simulink model "StarshipSystemModel"  (R2025b)
settings: Solver=VariableStepAuto  StartTime=0.0  StopTime=10.0  RelTol=1e-3
model workspace (MAT data in the model file):
  ActiveGNCMode = Simulink.Bus
  ActiveGNCMode.Alignment = -1
  ActiveGNCMode.PreserveElementDimensions = 0
  ActiveGNCMode.Elements_internal(1) = Simulink.BusElement
  ActiveGNCMode.Elements_internal(1).DimensionsMode = 'Fixed'
  ActiveGNCMode.Elements_internal(1).SamplingMode = 'Sample based'
  ActiveGNCMode.Elements_internal(1).SampleTime = -1
  ActiveGNCMode.Elements_internal(1).Name = 'stageID'
  ActiveGNCMode.Elements_internal(1).DataType_internal = 'uint8'
  ActiveGNCMode.Elements_internal(1).Complexity = 'real'
  ActiveGNCMode.Elements_internal(1).Dimensions = 1
  ActiveGNCMode.Elements_internal(2) = Simulink.BusElement
  ActiveGNCMode.Elements_internal(2).DimensionsMode = 'Fixed'
  ActiveGNCMode.Elements_internal(2).SamplingMode = 'Sample based'
  ActiveGNCMode.Elements_internal(2).SampleTime = -1
  ActiveGNCMode.Elements_internal(2).Name = 'phaseID'
  ActiveGNCMode.Elements_internal(2).DataType_internal = 'uint8'
  ActiveGNCMode.Elements_internal(2).Complexity = 'real'
  ActiveGNCMode.Elements_internal(2).Dimensions = 1
  ActiveGNCMode.Elements_internal(3) = Simulink.BusElement
  ActiveGNCMode.Elements_internal(3).DimensionsMode = 'Fixed'
  ActiveGNCMode.Elements_internal(3).SamplingMode = 'Sample based'
  ActiveGNCMode.Elements_internal(3).SampleTime = -1
  ActiveGNCMode.Elements_internal(3).Name = 'modeID'
  ActiveGNCMode.Elements_internal(3).DataType_internal = 'uint16'
  ActiveGNCMode.Elements_internal(3).Complexity = 'real'
  ActiveGNCMode.Elements_internal(3).Dimensions = 1
  ActiveGNCMode.Elements_internal(4) = Simulink.BusElement
  ActiveGNCMode.Elements_internal(4).DimensionsMode = 'Fixed'
  ActiveGNCMode.Elements_internal(4).SamplingMode = 'Sample based'
  ActiveGNCMode.Elements_internal(4).SampleTime = -1
  ActiveGNCMode.Elements_internal(4).DocUnits = 's'
  ActiveGNCMode.Elements_internal(4).Name = 'timestamp'
  ActiveGNCMode.Elements_internal(4).DataType_internal = 'double'
  ActiveGNCMode.Elements_internal(4).Complexity = 'real'
  ActiveGNCMode.Elements_internal(4).Dimensions = 1
  ActiveGNCMode.DataScope = 'Auto'
  AerodynamicControlCommand = Simulink.Bus
  AerodynamicControlCommand.Alignment = -1
  AerodynamicControlCommand.PreserveElementDimensions = 0
  AerodynamicControlCommand.Elements_internal(1) = Simulink.BusElement
  AerodynamicControlCommand.Elements_internal(1).DimensionsMode = 'Fixed'
  AerodynamicControlCommand.Elements_internal(1).SamplingMode = 'Sample based'
  AerodynamicControlCommand.Elements_internal(1).SampleTime = -1
  AerodynamicControlCommand.Elements_internal(1).DocUnits = 'rad'
  AerodynamicControlCommand.Elements_internal(1).Name = 'surfaceCommand'
  AerodynamicControlCommand.Elements_internal(1).DataType_internal = 'double'
  AerodynamicControlCommand.Elements_internal(1).Complexity = 'real'
  AerodynamicControlCommand.Elements_internal(1).Dimensions = 1
  AerodynamicControlCommand.Elements_internal(2) = Simulink.BusElement
  AerodynamicControlCommand.Elements_internal(2).DimensionsMode = 'Fixed'
  AerodynamicControlCommand.Elements_internal(2).SamplingMode = 'Sample based'
  AerodynamicControlCommand.Elements_internal(2).SampleTime = -1
  AerodynamicControlCommand.Elements_internal(2).Name = 'mode'
  AerodynamicControlCommand.Elements_internal(2).DataType_internal = 'enum'
  AerodynamicControlCommand.Elements_internal(2).Complexity = 'real'
  AerodynamicControlCommand.Elements_internal(2).Dimensions = 1
  AerodynamicControlCommand.Elements_internal(3) = Simulink.BusElement
  AerodynamicControlCommand.Elements_internal(3).DimensionsMode = 'Fixed'
  AerodynamicControlCommand.Elements_internal(3).SamplingMode = 'Sample based'
  AerodynamicControlCommand.Elements_internal(3).SampleTime = -1
  AerodynamicControlCommand.Elements_internal(3).Name = 'enable'
  AerodynamicControlCommand.Elements_internal(3).DataType_internal = 'boolean'
  AerodynamicControlCommand.Elements_internal(3).Complexity = 'real'
  AerodynamicControlCommand.Elements_internal(3).Dimensions = 1
  AerodynamicControlCommand.Elements_internal(4) = Simulink.BusElement
  AerodynamicControlCommand.Elements_internal(4).DimensionsMode = 'Fixed'
  AerodynamicControlCommand.Elements_internal(4).SamplingMode = 'Sample based'
  AerodynamicControlCommand.Elements_internal(4).SampleTime = -1
  AerodynamicControlCommand.Elements_internal(4).Name = 'validity'
  AerodynamicControlCommand.Elements_internal(4).DataType_internal = 'enum'
  AerodynamicControlCommand.Elements_internal(4).Complexity = 'real'
  AerodynamicControlCommand.Elements_internal(4).Dimensions = 1
  AerodynamicControlCommand.Elements_internal(5) = Simulink.BusElement
  AerodynamicControlCommand.Elements_internal(5).DimensionsMode = 'Fixed'
  AerodynamicControlCommand.Elements_internal(5).SamplingMode = 'Sample based'
  AerodynamicControlCommand.Elements_internal(5).SampleTime = -1
  AerodynamicControlCommand.Elements_internal(5).DocUnits = 's'
  AerodynamicControlCommand.Elements_internal(5).Name = 'timestamp'
  AerodynamicControlCommand.Elements_internal(5).DataType_internal = 'double'
  AerodynamicControlCommand.Elements_internal(5).Complexity = 'real'
  AerodynamicControlCommand.Elements_internal(5).Dimensions = 1
  AerodynamicControlCommand.DataScope = 'Auto'
  AerodynamicLoad = Simulink.Bus
  AerodynamicLoad.Alignment = -1
  AerodynamicLoad.PreserveElementDimensions = 0
  AerodynamicLoad.Elements_internal(1) = Simulink.BusElement
  AerodynamicLoad.Elements_internal(1).DimensionsMode = 'Fixed'
  AerodynamicLoad.Elements_internal(1).SamplingMode = 'Sample based'
  AerodynamicLoad.Elements_internal(1).SampleTime = -1
  AerodynamicLoad.Elements_internal(1).DocUnits = 'N'
  AerodynamicLoad.Elements_internal(1).Name = 'force'
  AerodynamicLoad.Elements_internal(1).DataType_internal = 'double'
  AerodynamicLoad.Elements_internal(1).Complexity = 'real'
  AerodynamicLoad.Elements_internal(1).Dimensions = 1
  AerodynamicLoad.Elements_internal(2) = Simulink.BusElement
  AerodynamicLoad.Elements_internal(2).DimensionsMode = 'Fixed'
  AerodynamicLoad.Elements_internal(2).SamplingMode = 'Sample based'
  AerodynamicLoad.Elements_internal(2).SampleTime = -1
  AerodynamicLoad.Elements_internal(2).DocUnits = 'N·m'
  AerodynamicLoad.Elements_internal(2).Name = 'moment'
  AerodynamicLoad.Elements_internal(2).DataType_internal = 'double'
  AerodynamicLoad.Elements_internal(2).Complexity = 'real'
  AerodynamicLoad.Elements_internal(2).Dimensions = 1
  AerodynamicLoad.Elements_internal(3) = Simulink.BusElement
  AerodynamicLoad.Elements_internal(3).DimensionsMode = 'Fixed'
  AerodynamicLoad.Elements_internal(3).SamplingMode = 'Sample based'
  AerodynamicLoad.Elements_internal(3).SampleTime = -1
  AerodynamicLoad.Elements_internal(3).Name = 'referenceFrame'
  AerodynamicLoad.Elements_internal(3).DataType_internal = 'string'
  AerodynamicLoad.Elements_internal(3).Complexity = 'real'
  AerodynamicLoad.Elements_internal(3).Dimensions = 1
  AerodynamicLoad.Elements_internal(4) = Simulink.BusElement
  AerodynamicLoad.Elements_internal(4).DimensionsMode = 'Fixed'
  AerodynamicLoad.Elements_internal(4).SamplingMode = 'Sample based'
  AerodynamicLoad.Elements_internal(4).SampleTime = -1
  AerodynamicLoad.Elements_internal(4).DocUnits = 'Pa'
  AerodynamicLoad.Elements_internal(4).Name = 'surfacePressure'
  AerodynamicLoad.Elements_internal(4).DataType_internal = 'double'
  AerodynamicLoad.Elements_internal(4).Complexity = 'real'
  AerodynamicLoad.Elements_internal(4).Dimensions = 1
  AerodynamicLoad.Elements_internal(5) = Simulink.BusElement
  AerodynamicLoad.Elements_internal(5).DimensionsMode = 'Fixed'
  AerodynamicLoad.Elements_internal(5).SamplingMode = 'Sample based'
  AerodynamicLoad.Elements_internal(5).SampleTime = -1
  AerodynamicLoad.Elements_internal(5).Name = 'validity'
  AerodynamicLoad.Elements_internal(5).DataType_internal = 'enum'
  AerodynamicLoad.Elements_internal(5).Complexity = 'real'
  AerodynamicLoad.Elements_internal(5).Dimensions = 1
  AerodynamicLoad.DataScope = 'Auto'
  AggregatedStream = Simulink.Bus
  AggregatedStream.Alignment = -1
  AggregatedStream.PreserveElementDimensions = 0
  AggregatedStream.Elements_internal(1) = Simulink.BusElement
  AggregatedStream.Elements_internal(1).DimensionsMode = 'Fixed'
  AggregatedStream.Elements_internal(1).SamplingMode = 'Sample based'
  AggregatedStream.Elements_internal(1).SampleTime = -1
  AggregatedStream.Elements_internal(1).Name = 'payload'
  AggregatedStream.Elements_internal(1).DataType_internal = 'uint8'
  AggregatedStream.Elements_internal(1).Complexity = 'real'
  AggregatedStream.Elements_internal(1).Dimensions = 1
  AggregatedStream.Elements_internal(2) = Simulink.BusElement
  AggregatedStream.Elements_internal(2).DimensionsMode = 'Fixed'
  AggregatedStream.Elements_internal(2).SamplingMode = 'Sample based'
  AggregatedStream.Elements_internal(2).SampleTime = -1
  AggregatedStream.Elements_internal(2).Name = 'sourceMix'
  AggregatedStream.Elements_internal(2).DataType_internal = 'double'
  AggregatedStream.Elements_internal(2).Complexity = 'real'
  AggregatedStream.Elements_internal(2).Dimensions = 1
  AggregatedStream.Elements_internal(3) = Simulink.BusElement
  AggregatedStream.Elements_internal(3).DimensionsMode = 'Fixed'
  AggregatedStream.Elements_internal(3).SamplingMode = 'Sample based'
  AggregatedStream.Elements_internal(3).SampleTime = -1
  AggregatedStream.Elements_internal(3).DocUnits = 's'
  AggregatedStream.Elements_internal(3).Name = 'timestamp'
  AggregatedStream.Elements_internal(3).DataType_internal = 'double'
  AggregatedStream.Elements_internal(3).Complexity = 'real'
  AggregatedStream.Elements_internal(3).Dimensions = 1
  AggregatedStream.DataScope = 'Auto'
  AllocatedEffectorDemand = Simulink.Bus
  AllocatedEffectorDemand.Alignment = -1
  AllocatedEffectorDemand.PreserveElementDimensions = 0
  AllocatedEffectorDemand.Elements_internal(1) = Simulink.BusElement
  AllocatedEffectorDemand.Elements_internal(1).DimensionsMode = 'Fixed'
  AllocatedEffectorDemand.Elements_internal(1).SamplingMode = 'Sample based'
  AllocatedEffectorDemand.Elements_internal(1).SampleTime = -1
  AllocatedEffectorDemand.Elements_internal(1).Name = 'effectorID'
  AllocatedEffectorDemand.Elements_internal(1).DataType_internal = 'uint16'
  AllocatedEffectorDemand.Elements_internal(1).Complexity = 'real'
  AllocatedEffectorDemand.Elements_internal(1).Dimensions = 1
  AllocatedEffectorDemand.Elements_internal(2) = Simulink.BusElement
  AllocatedEffectorDemand.Elements_internal(2).DimensionsMode = 'Fixed'
  AllocatedEffectorDemand.Elements_internal(2).SamplingMode = 'Sample based'
  AllocatedEffectorDemand.Elements_internal(2).SampleTime = -1
  AllocatedEffectorDemand.Elements_internal(2).Name = 'demand'
  AllocatedEffectorDemand.Elements_internal(2).DataType_internal = 'double'
  AllocatedEffectorDemand.Elements_internal(2).Complexity = 'real'
  AllocatedEffectorDemand.Elements_internal(2).Dimensions = 1
  AllocatedEffectorDemand.Elements_internal(3) = Simulink.BusElement
  AllocatedEffectorDemand.Elements_internal(3).DimensionsMode = 'Fixed'
  AllocatedEffectorDemand.Elements_internal(3).SamplingMode = 'Sample based'
  AllocatedEffectorDemand.Elements_internal(3).SampleTime = -1
  AllocatedEffectorDemand.Elements_internal(3).Name = 'validity'
  AllocatedEffectorDemand.Elements_internal(3).DataType_internal = 'uint8'
  AllocatedEffectorDemand.Elements_internal(3).Complexity = 'real'
  AllocatedEffectorDemand.Elements_internal(3).Dimensions = 1
  AllocatedEffectorDemand.Elements_internal(4) = Simulink.BusElement
  AllocatedEffectorDemand.Elements_internal(4).DimensionsMode = 'Fixed'
  AllocatedEffectorDemand.Elements_internal(4).SamplingMode = 'Sample based'
  AllocatedEffectorDemand.Elements_internal(4).SampleTime = -1
  AllocatedEffectorDemand.Elements_internal(4).DocUnits = 's'
  AllocatedEffectorDemand.Elements_internal(4).Name = 'timestamp'
  AllocatedEffectorDemand.Elements_internal(4).DataType_internal = 'double'
  AllocatedEffectorDemand.Elements_internal(4).Complexity = 'real'
  AllocatedEffectorDemand.Elements_internal(4).Dimensions = 1
  AllocatedEffectorDemand.DataScope = 'Auto'
  AttitudeControlDemand = Simulink.Bus
  AttitudeControlDemand.Alignment = -1
  AttitudeControlDemand.PreserveElementDimensions = 0
  AttitudeControlDemand.Elements_internal(1) = Simulink.BusElement
  AttitudeControlDemand.Elements_internal(1).DimensionsMode = 'Fixed'
  AttitudeControlDemand.Elements_internal(1).SamplingMode = 'Sample based'
  AttitudeControlDemand.Elements_internal(1).SampleTime = -1
  AttitudeControlDemand.Elements_internal(1).DocUnits = 'N.m'
  AttitudeControlDemand.Elements_internal(1).Name = 'torqueDemand'
  AttitudeControlDemand.Elements_internal(1).DataType_internal = 'double'
  AttitudeControlDemand.Elements_internal(1).Complexity = 'real'
  AttitudeControlDemand.Elements_internal(1).Dimensions = 3
  AttitudeControlDemand.Elements_internal(2) = Simulink.BusElement
  AttitudeControlDemand.Elements_internal(2).DimensionsMode = 'Fixed'
  AttitudeControlDemand.Elements_internal(2).SamplingMode = 'Sample based'
  AttitudeControlDemand.Elements_internal(2).SampleTime = -1
  AttitudeControlDemand.Elements_internal(2).DocUnits = 's'
  AttitudeControlDemand.Elements_internal(2).Name = 'timestamp'
  AttitudeControlDemand.Elements_internal(2).DataType_internal = 'double'
  AttitudeControlDemand.Elements_internal(2).Complexity = 'real'
  AttitudeControlDemand.Elements_internal(2).Dimensions = 1
  AttitudeControlDemand.DataScope = 'Auto'
  AttitudeGuidanceCommand = Simulink.Bus
  AttitudeGuidanceCommand.Alignment = -1
  AttitudeGuidanceCommand.PreserveElementDimensions = 0
  AttitudeGuidanceCommand.Elements_internal(1) = Simulink.BusElement
  AttitudeGuidanceCommand.Elements_internal(1).DimensionsMode = 'Fixed'
  AttitudeGuidanceCommand.Elements_internal(1).SamplingMode = 'Sample based'
  AttitudeGuidanceCommand.Elements_internal(1).SampleTime = -1
  AttitudeGuidanceCommand.Elements_internal(1).Name = 'attitudeTarget'
  AttitudeGuidanceCommand.Elements_internal(1).DataType_internal = 'double'
  AttitudeGuidanceCommand.Elements_internal(1).Complexity = 'real'
  AttitudeGuidanceCommand.Elements_internal(1).Dimensions = 4
  AttitudeGuidanceCommand.Elements_internal(2) = Simulink.BusElement
  AttitudeGuidanceCommand.Elements_internal(2).DimensionsMode = 'Fixed'
  AttitudeGuidanceCommand.Elements_internal(2).SamplingMode = 'Sample based'
  AttitudeGuidanceCommand.Elements_internal(2).SampleTime = -1
  AttitudeGuidanceCommand.Elements_internal(2).Name = 'rateTarget'
  AttitudeGuidanceCommand.Elements_internal(2).DataType_internal = 'double'
  AttitudeGuidanceCommand.Elements_internal(2).Complexity = 'real'
  AttitudeGuidanceCommand.Elements_internal(2).Dimensions = 3
  AttitudeGuidanceCommand.Elements_internal(3) = Simulink.BusElement
  AttitudeGuidanceCommand.Elements_internal(3).DimensionsMode = 'Fixed'
  AttitudeGuidanceCommand.Elements_internal(3).SamplingMode = 'Sample based'
  AttitudeGuidanceCommand.Elements_internal(3).SampleTime = -1
  AttitudeGuidanceCommand.Elements_internal(3).DocUnits = 's'
  AttitudeGuidanceCommand.Elements_internal(3).Name = 'timestamp'
  AttitudeGuidanceCommand.Elements_internal(3).DataType_internal = 'double'
  AttitudeGuidanceCommand.Elements_internal(3).Complexity = 'real'
  AttitudeGuidanceCommand.Elements_internal(3).Dimensions = 1
  AttitudeGuidanceCommand.DataScope = 'Auto'
  AttitudeRateState = Simulink.Bus
  AttitudeRateState.Alignment = -1
  AttitudeRateState.PreserveElementDimensions = 0
  AttitudeRateState.Elements_internal(1) = Simulink.BusElement
  AttitudeRateState.Elements_internal(1).DimensionsMode = 'Fixed'
  AttitudeRateState.Elements_internal(1).SamplingMode = 'Sample based'
  AttitudeRateState.Elements_internal(1).SampleTime = -1
  AttitudeRateState.Elements_internal(1).Name = 'attitude'
  AttitudeRateState.Elements_internal(1).DataType_internal = 'double'
  AttitudeRateState.Elements_internal(1).Complexity = 'real'
  AttitudeRateState.Elements_internal(1).Dimensions = 4
  AttitudeRateState.Elements_internal(2) = Simulink.BusElement
  AttitudeRateState.Elements_internal(2).DimensionsMode = 'Fixed'
  AttitudeRateState.Elements_internal(2).SamplingMode = 'Sample based'
  AttitudeRateState.Elements_internal(2).SampleTime = -1
  AttitudeRateState.Elements_internal(2).DocUnits = 'rad/s'
  AttitudeRateState.Elements_internal(2).Name = 'angularRate'
  AttitudeRateState.Elements_internal(2).DataType_internal = 'double'
  AttitudeRateState.Elements_internal(2).Complexity = 'real'
  AttitudeRateState.Elements_internal(2).Dimensions = 3
  AttitudeRateState.Elements_internal(3) = Simulink.BusElement
  AttitudeRateState.Elements_internal(3).DimensionsMode = 'Fixed'
  AttitudeRateState.Elements_internal(3).SamplingMode = 'Sample based'
  AttitudeRateState.Elements_internal(3).SampleTime = -1
  AttitudeRateState.Elements_internal(3).DocUnits = 's'
  AttitudeRateState.Elements_internal(3).Name = 'timestamp'
  AttitudeRateState.Elements_internal(3).DataType_internal = 'double'
  AttitudeRateState.Elements_internal(3).Complexity = 'real'
  AttitudeRateState.Elements_internal(3).Dimensions = 1
  AttitudeRateState.DataScope = 'Auto'
  AutogenousPressurantGas = Simulink.ConnectionBus
  AutogenousPressurantGas.Elements_internal = Simulink.ConnectionElement
  AutogenousPressurantGas.Elements_internal.Name = 'Element'
  AutogenousPressurantGas.Elements_internal.Type_internal = 'Connection: foundation.gas.gas'
  CandidateFaultIndication = Simulink.Bus
  CandidateFaultIndication.Alignment = -1
  CandidateFaultIndication.PreserveElementDimensions = 0
  CandidateFaultIndication.Elements_internal(1) = Simulink.BusElement
  CandidateFaultIndication.Elements_internal(1).DimensionsMode = 'Fixed'
  CandidateFaultIndication.Elements_internal(1).SamplingMode = 'Sample based'
  CandidateFaultIndication.Elements_internal(1).SampleTime = -1
  CandidateFaultIndication.Elements_internal(1).Name = 'faultCode'
  CandidateFaultIndication.Elements_internal(1).DataType_internal = 'string'
  CandidateFaultIndication.Elements_internal(1).Complexity = 'real'
  CandidateFaultIndication.Elements_internal(1).Dimensions = 1
  CandidateFaultIndication.Elements_internal(2) = Simulink.BusElement
  CandidateFaultIndication.Elements_internal(2).DimensionsMode = 'Fixed'
  CandidateFaultIndication.Elements_internal(2).SamplingMode = 'Sample based'
  CandidateFaultIndication.Elements_internal(2).SampleTime = -1
  CandidateFaultIndication.Elements_internal(2).Name = 'confidence'
  CandidateFaultIndication.Elements_internal(2).DataType_internal = 'string'
  CandidateFaultIndication.Elements_internal(2).Complexity = 'real'
  CandidateFaultIndication.Elements_internal(2).Dimensions = 1
  CandidateFaultIndication.DataScope = 'Auto'
  CombustionGasFeed = Simulink.ConnectionBus
  CombustionGasFeed.Elements_internal = Simulink.ConnectionElement
  CombustionGasFeed.Elements_internal.Name = 'Element'
  CombustionGasFeed.Elements_internal.Type_internal = 'Connection: foundation.gas.gas'
  CommandPathHealth = Simulink.Bus
  CommandPathHealth.Alignment = -1
  CommandPathHealth.PreserveElementDimensions = 0
  CommandPathHealth.Elements_internal(1) = Simulink.BusElement
  CommandPathHealth.Elements_internal(1).DimensionsMode = 'Fixed'
  CommandPathHealth.Elements_internal(1).SamplingMode = 'Sample based'
  CommandPathHealth.Elements_internal(1).SampleTime = -1
  CommandPathHealth.Elements_internal(1).Name = 'availability'
  CommandPathHealth.Elements_internal(1).DataType_internal = 'uint8'
  CommandPathHealth.Elements_internal(1).Complexity = 'real'
  CommandPathHealth.Elements_internal(1).Dimensions = 1
  CommandPathHealth.Elements_internal(2) = Simulink.BusElement
  CommandPathHealth.Elements_internal(2).DimensionsMode = 'Fixed'
  CommandPathHealth.Elements_internal(2).SamplingMode = 'Sample based'
  CommandPathHealth.Elements_internal(2).SampleTime = -1
  CommandPathHealth.Elements_internal(2).Name = 'inhibitedReason'
  CommandPathHealth.Elements_internal(2).DataType_internal = 'uint16'
  CommandPathHealth.Elements_internal(2).Complexity = 'real'
  CommandPathHealth.Elements_internal(2).Dimensions = 1
  CommandPathHealth.Elements_internal(3) = Simulink.BusElement
  CommandPathHealth.Elements_internal(3).DimensionsMode = 'Fixed'
  CommandPathHealth.Elements_internal(3).SamplingMode = 'Sample based'
  CommandPathHealth.Elements_internal(3).SampleTime = -1
  CommandPathHealth.Elements_internal(3).DocUnits = 's'
  CommandPathHealth.Elements_internal(3).Name = 'timestamp'
  CommandPathHealth.Elements_internal(3).DataType_internal = 'double'
  CommandPathHealth.Elements_internal(3).Complexity = 'real'
  CommandPathHealth.Elements_internal(3).Dimensions = 1
  CommandPathHealth.DataScope = 'Auto'
  ControlMode = Simulink.ValueType
  ControlMode.DataType = 'enum'
  DownlinkSignal = Simulink.Bus
  DownlinkSignal.Alignment = -1
  DownlinkSignal.PreserveElementDimensions = 0
  DownlinkSignal.Elements_internal(1) = Simulink.BusElement
  DownlinkSignal.Elements_internal(1).DimensionsMode = 'Fixed'
  DownlinkSignal.Elements_internal(1).SamplingMode = 'Sample based'
  DownlinkSignal.Elements_internal(1).SampleTime = -1
  DownlinkSignal.Elements_internal(1).Name = 'payload'
  DownlinkSignal.Elements_internal(1).DataType_internal = 'uint8'
  DownlinkSignal.Elements_internal(1).Complexity = 'real'
  DownlinkSignal.Elements_internal(1).Dimensions = 1
  DownlinkSignal.Elements_internal(2) = Simulink.BusElement
  DownlinkSignal.Elements_internal(2).DimensionsMode = 'Fixed'
  DownlinkSignal.Elements_internal(2).SamplingMode = 'Sample based'
  DownlinkSignal.Elements_internal(2).SampleTime = -1
  DownlinkSignal.Elements_internal(2).Description = '{Relay, DirectRF}'
  DownlinkSignal.Elements_internal(2).Name = 'pathUsed'
  DownlinkSignal.Elements_internal(2).DataType_internal = 'enumration'
  DownlinkSignal.Elements_internal(2).Complexity = 'real'
  DownlinkSignal.Elements_internal(2).Dimensions = 1
  DownlinkSignal.Elements_internal(3) = Simulink.BusElement
  DownlinkSignal.Elements_internal(3).DimensionsMode = 'Fixed'
  DownlinkSignal.Elements_internal(3).SamplingMode = 'Sample based'
  DownlinkSignal.Elements_internal(3).SampleTime = -1
  DownlinkSignal.Elements_internal(3).DocUnits = 's'
  DownlinkSignal.Elements_internal(3).Name = 'timestamp'
  DownlinkSignal.Elements_internal(3).DataType_internal = 'double'
  DownlinkSignal.Elements_internal(3).Complexity = 'real'
  DownlinkSignal.Elements_internal(3).Dimensions = 1
  DownlinkSignal.DataScope = 'Auto'
  ElectricalPower = Simulink.ConnectionBus
  ElectricalPower.Elements_internal = Simulink.ConnectionElement
  ElectricalPower.Elements_internal.Name = 'Element'
  ElectricalPower.Elements_internal.Type_internal = 'Connection: foundation.electrical.electrical'
  EngineTelemetry = Simulink.Bus
  EngineTelemetry.Alignment = -1
  EngineTelemetry.PreserveElementDimensions = 0
  EngineTelemetry.Elements_internal(1) = Simulink.BusElement
  EngineTelemetry.Elements_internal(1).DimensionsMode = 'Fixed'
  EngineTelemetry.Elements_internal(1).SamplingMode = 'Sample based'
  EngineTelemetry.Elements_internal(1).SampleTime = -1
  EngineTelemetry.Elements_internal(1).DocUnits = 'Pa'
  EngineTelemetry.Elements_internal(1).Name = 'chamberPressure'
  EngineTelemetry.Elements_internal(1).DataType_internal = 'double'
  EngineTelemetry.Elements_internal(1).Complexity = 'real'
  EngineTelemetry.Elements_internal(1).Dimensions = 1
  EngineTelemetry.Elements_internal(2) = Simulink.BusElement
  EngineTelemetry.Elements_internal(2).DimensionsMode = 'Fixed'
  EngineTelemetry.Elements_internal(2).SamplingMode = 'Sample based'
  EngineTelemetry.Elements_internal(2).SampleTime = -1
  EngineTelemetry.Elements_internal(2).DocUnits = 'rpm'
  EngineTelemetry.Elements_internal(2).Name = 'turbopumpSpeed'
  EngineTelemetry.Elements_internal(2).DataType_internal = 'double'
  EngineTelemetry.Elements_internal(2).Complexity = 'real'
  EngineTelemetry.Elements_internal(2).Dimensions = 1
  EngineTelemetry.Elements_internal(3) = Simulink.BusElement
  EngineTelemetry.Elements_internal(3).DimensionsMode = 'Fixed'
  EngineTelemetry.Elements_internal(3).SamplingMode = 'Sample based'
  EngineTelemetry.Elements_internal(3).SampleTime = -1
  EngineTelemetry.Elements_internal(3).DocUnits = 'K'
  EngineTelemetry.Elements_internal(3).Name = 'temperature'
  EngineTelemetry.Elements_internal(3).DataType_internal = 'double'
  EngineTelemetry.Elements_internal(3).Complexity = 'real'
  EngineTelemetry.Elements_internal(3).Dimensions = 1
  EngineTelemetry.Elements_internal(4) = Simulink.BusElement
  EngineTelemetry.Elements_internal(4).DimensionsMode = 'Fixed'
  EngineTelemetry.Elements_internal(4).SamplingMode = 'Sample based'
  EngineTelemetry.Elements_internal(4).SampleTime = -1
  EngineTelemetry.Elements_internal(4).Name = 'status'
  EngineTelemetry.Elements_internal(4).DataType_internal = 'uint8'
  EngineTelemetry.Elements_internal(4).Complexity = 'real'
  EngineTelemetry.Elements_internal(4).Dimensions = 1
  EngineTelemetry.DataScope = 'Auto'
  ExecutionContext = Simulink.Bus
  ExecutionContext.Alignment = -1
  ExecutionContext.PreserveElementDimensions = 0
  ExecutionContext.Elements_internal(1) = Simulink.BusElement
  ExecutionContext.Elements_internal(1).DimensionsMode = 'Fixed'
  ExecutionContext.Elements_internal(1).SamplingMode = 'Sample based'
  ExecutionContext.Elements_internal(1).SampleTime = -1
  ExecutionContext.Elements_internal(1).Name = 'cycleID'
  ExecutionContext.Elements_internal(1).DataType_internal = 'uint32'
  ExecutionContext.Elements_internal(1).Complexity = 'real'
  ExecutionContext.Elements_internal(1).Dimensions = 1
  ExecutionContext.Elements_internal(2) = Simulink.BusElement
  ExecutionContext.Elements_internal(2).DimensionsMode = 'Fixed'
  ExecutionContext.Elements_internal(2).SamplingMode = 'Sample based'
  ExecutionContext.Elements_internal(2).SampleTime = -1
  ExecutionContext.Elements_internal(2).Name = 'phaseID'
  ExecutionContext.Elements_internal(2).DataType_internal = 'uint8'
  ExecutionContext.Elements_internal(2).Complexity = 'real'
  ExecutionContext.Elements_internal(2).Dimensions = 1
  ExecutionContext.Elements_internal(3) = Simulink.BusElement
  ExecutionContext.Elements_internal(3).DimensionsMode = 'Fixed'
  ExecutionContext.Elements_internal(3).SamplingMode = 'Sample based'
  ExecutionContext.Elements_internal(3).SampleTime = -1
  ExecutionContext.Elements_internal(3).Name = 'executionStatus'
  ExecutionContext.Elements_internal(3).DataType_internal = 'uint8'
  ExecutionContext.Elements_internal(3).Complexity = 'real'
  ExecutionContext.Elements_internal(3).Dimensions = 1
  ExecutionContext.Elements_internal(4) = Simulink.BusElement
  ExecutionContext.Elements_internal(4).DimensionsMode = 'Fixed'
  ExecutionContext.Elements_internal(4).SamplingMode = 'Sample based'
  ExecutionContext.Elements_internal(4).SampleTime = -1
  ExecutionContext.Elements_internal(4).DocUnits = 's'
  ExecutionContext.Elements_internal(4).Name = 'timestamp'
  ExecutionContext.Elements_internal(4).DataType_internal = 'double'
  ExecutionContext.Elements_internal(4).Complexity = 'real'
  ExecutionContext.Elements_internal(4).Dimensions = 1
  ExecutionContext.DataScope = 'Auto'
  FaultDiagnosisResult = Simulink.Bus
  FaultDiagnosisResult.Alignment = -1
  FaultDiagnosisResult.PreserveElementDimensions = 0
  FaultDiagnosisResult.Elements_internal(1) = Simulink.BusElement
  FaultDiagnosisResult.Elements_internal(1).DimensionsMode = 'Fixed'
  FaultDiagnosisResult.Elements_internal(1).SamplingMode = 'Sample based'
  FaultDiagnosisResult.Elements_internal(1).SampleTime = -1
  FaultDiagnosisResult.Elements_internal(1).Name = 'faultCode'
  FaultDiagnosisResult.Elements_internal(1).DataType_internal = 'string'
  FaultDiagnosisResult.Elements_internal(1).Complexity = 'real'
  FaultDiagnosisResult.Elements_internal(1).Dimensions = 1
  FaultDiagnosisResult.Elements_internal(2) = Simulink.BusElement
  FaultDiagnosisResult.Elements_internal(2).DimensionsMode = 'Fixed'
  FaultDiagnosisResult.Elements_internal(2).SamplingMode = 'Sample based'
  FaultDiagnosisResult.Elements_internal(2).SampleTime = -1
  FaultDiagnosisResult.Elements_internal(2).Name = 'confidence'
  FaultDiagnosisResult.Elements_internal(2).DataType_internal = 'string'
  FaultDiagnosisResult.Elements_internal(2).Complexity = 'real'
  FaultDiagnosisResult.Elements_internal(2).Dimensions = 1
  FaultDiagnosisResult.DataScope = 'Auto'
  GNCDataContext = Simulink.Bus
  GNCDataContext.Alignment = -1
  GNCDataContext.PreserveElementDimensions = 0
  GNCDataContext.Elements_internal(1) = Simulink.BusElement
  GNCDataContext.Elements_internal(1).DimensionsMode = 'Fixed'
  GNCDataContext.Elements_internal(1).SamplingMode = 'Sample based'
  GNCDataContext.Elements_internal(1).SampleTime = -1
  GNCDataContext.Elements_internal(1).Name = 'sourceID'
  GNCDataContext.Elements_internal(1).DataType_internal = 'uint16'
  GNCDataContext.Elements_internal(1).Complexity = 'real'
  GNCDataContext.Elements_internal(1).Dimensions = 1
  GNCDataContext.Elements_internal(2) = Simulink.BusElement
  GNCDataContext.Elements_internal(2).DimensionsMode = 'Fixed'
  GNCDataContext.Elements_internal(2).SamplingMode = 'Sample based'
  GNCDataContext.Elements_internal(2).SampleTime = -1
  GNCDataContext.Elements_internal(2).Name = 'dataClass'
  GNCDataContext.Elements_internal(2).DataType_internal = 'uint8'
  GNCDataContext.Elements_internal(2).Complexity = 'real'
  GNCDataContext.Elements_internal(2).Dimensions = 1
  GNCDataContext.Elements_internal(3) = Simulink.BusElement
  GNCDataContext.Elements_internal(3).DimensionsMode = 'Fixed'
  GNCDataContext.Elements_internal(3).SamplingMode = 'Sample based'
  GNCDataContext.Elements_internal(3).SampleTime = -1
  GNCDataContext.Elements_internal(3).DocUnits = 's'
  GNCDataContext.Elements_internal(3).Name = 'timestamp'
  GNCDataContext.Elements_internal(3).DataType_internal = 'double'
  GNCDataContext.Elements_internal(3).Complexity = 'real'
  GNCDataContext.Elements_internal(3).Dimensions = 1
  GNCDataContext.Elements_internal(4) = Simulink.BusElement
  GNCDataContext.Elements_internal(4).DimensionsMode = 'Fixed'
  GNCDataContext.Elements_internal(4).SamplingMode = 'Sample based'
  GNCDataContext.Elements_internal(4).SampleTime = -1
  GNCDataContext.Elements_internal(4).Name = 'validity'
  GNCDataContext.Elements_internal(4).DataType_internal = 'uint8'
  GNCDataContext.Elements_internal(4).Complexity = 'real'
  GNCDataContext.Elements_internal(4).Dimensions = 1
  GNCDataContext.DataScope = 'Auto'
  GNCHealthState = Simulink.Bus
  GNCHealthState.Alignment = -1
  GNCHealthState.PreserveElementDimensions = 0
  GNCHealthState.Elements_internal(1) = Simulink.BusElement
  GNCHealthState.Elements_internal(1).DimensionsMode = 'Fixed'
  GNCHealthState.Elements_internal(1).SamplingMode = 'Sample based'
  GNCHealthState.Elements_internal(1).SampleTime = -1
  GNCHealthState.Elements_internal(1).Name = 'healthState'
  GNCHealthState.Elements_internal(1).DataType_internal = 'uint8'
  GNCHealthState.Elements_internal(1).Complexity = 'real'
  GNCHealthState.Elements_internal(1).Dimensions = 1
  GNCHealthState.Elements_internal(2) = Simulink.BusElement
  GNCHealthState.Elements_internal(2).DimensionsMode = 'Fixed'
  GNCHealthState.Elements_internal(2).SamplingMode = 'Sample based'
  GNCHealthState.Elements_internal(2).SampleTime = -1
  GNCHealthState.Elements_internal(2).Name = 'faultCode'
  GNCHealthState.Elements_internal(2).DataType_internal = 'uint16'
  GNCHealthState.Elements_internal(2).Complexity = 'real'
  GNCHealthState.Elements_internal(2).Dimensions = 1
  GNCHealthState.Elements_internal(3) = Simulink.BusElement
  GNCHealthState.Elements_internal(3).DimensionsMode = 'Fixed'
  GNCHealthState.Elements_internal(3).SamplingMode = 'Sample based'
  GNCHealthState.Elements_internal(3).SampleTime = -1
  GNCHealthState.Elements_internal(3).DocUnits = 's'
  GNCHealthState.Elements_internal(3).Name = 'timestamp'
  GNCHealthState.Elements_internal(3).DataType_internal = 'double'
  GNCHealthState.Elements_internal(3).Complexity = 'real'
  GNCHealthState.Elements_internal(3).Dimensions = 1
  GNCHealthState.DataScope = 'Auto'
  GNCStateEstimate = Simulink.Bus
  GNCStateEstimate.Alignment = -1
  GNCStateEstimate.PreserveElementDimensions = 0
  GNCStateEstimate.Elements_internal(1) = Simulink.BusElement
  GNCStateEstimate.Elements_internal(1).DimensionsMode = 'Fixed'
  GNCStateEstimate.Elements_internal(1).SamplingMode = 'Sample based'
  GNCStateEstimate.Elements_internal(1).SampleTime = -1
  GNCStateEstimate.Elements_internal(1).DocUnits = 'm'
  GNCStateEstimate.Elements_internal(1).Name = 'position'
  GNCStateEstimate.Elements_internal(1).DataType_internal = 'double'
  GNCStateEstimate.Elements_internal(1).Complexity = 'real'
  GNCStateEstimate.Elements_internal(1).Dimensions = 3
  GNCStateEstimate.Elements_internal(2) = Simulink.BusElement
  GNCStateEstimate.Elements_internal(2).DimensionsMode = 'Fixed'
  GNCStateEstimate.Elements_internal(2).SamplingMode = 'Sample based'
  GNCStateEstimate.Elements_internal(2).SampleTime = -1
  GNCStateEstimate.Elements_internal(2).DocUnits = 'm/s'
  GNCStateEstimate.Elements_internal(2).Name = 'velocity'
  GNCStateEstimate.Elements_internal(2).DataType_internal = 'double'
  GNCStateEstimate.Elements_internal(2).Complexity = 'real'
  GNCStateEstimate.Elements_internal(2).Dimensions = 3
  GNCStateEstimate.Elements_internal(3) = Simulink.BusElement
  GNCStateEstimate.Elements_internal(3).DimensionsMode = 'Fixed'
  GNCStateEstimate.Elements_internal(3).SamplingMode = 'Sample based'
  GNCStateEstimate.Elements_internal(3).SampleTime = -1
  GNCStateEstimate.Elements_internal(3).Name = 'attitude'
  GNCStateEstimate.Elements_internal(3).DataType_internal = 'double'
  GNCStateEstimate.Elements_internal(3).Complexity = 'real'
  GNCStateEstimate.Elements_internal(3).Dimensions = 4
  GNCStateEstimate.Elements_internal(4) = Simulink.BusElement
  GNCStateEstimate.Elements_internal(4).DimensionsMode = 'Fixed'
  GNCStateEstimate.Elements_internal(4).SamplingMode = 'Sample based'
  GNCStateEstimate.Elements_internal(4).SampleTime = -1
  GNCStateEstimate.Elements_internal(4).DocUnits = 'rad/s'
  GNCStateEstimate.Elements_internal(4).Name = 'angularRate'
  GNCStateEstimate.Elements_internal(4).DataType_internal = 'double'
  GNCStateEstimate.Elements_internal(4).Complexity = 'real'
  GNCStateEstimate.Elements_internal(4).Dimensions = 3
  GNCStateEstimate.Elements_internal(5) = Simulink.BusElement
  GNCStateEstimate.Elements_internal(5).DimensionsMode = 'Fixed'
  GNCStateEstimate.Elements_internal(5).SamplingMode = 'Sample based'
  GNCStateEstimate.Elements_internal(5).SampleTime = -1
  GNCStateEstimate.Elements_internal(5).DocUnits = 's'
  GNCStateEstimate.Elements_internal(5).Name = 'timestamp'
  GNCStateEstimate.Elements_internal(5).DataType_internal = 'double'
  GNCStateEstimate.Elements_internal(5).Complexity = 'real'
  GNCStateEstimate.Elements_internal(5).Dimensions = 1
  GNCStateEstimate.DataScope = 'Auto'
  GimbalAngle = Simulink.ValueType
  GimbalAngle.Min = -15
  GimbalAngle.Max = 15
  GimbalAngle.Unit = 'deg'
  GimbalMotion = Simulink.ConnectionBus
  GimbalMotion.Elements_internal = Simulink.ConnectionElement
  GimbalMotion.Elements_internal.Name = 'Element'
  GimbalMotion.Elements_internal.Type_internal = 'Connection: foundation.mechanical.rotational.rotational'
  GroundCheckoutLink = Simulink.Bus
  GroundCheckoutLink.Alignment = -1
  GroundCheckoutLink.PreserveElementDimensions = 0
  GroundCheckoutLink.Elements_internal(1) = Simulink.BusElement
  GroundCheckoutLink.Elements_internal(1).DimensionsMode = 'Fixed'
  GroundCheckoutLink.Elements_internal(1).SamplingMode = 'Sample based'
  GroundCheckoutLink.Elements_internal(1).SampleTime = -1
  GroundCheckoutLink.Elements_internal(1).Name = 'payload'
  GroundCheckoutLink.Elements_internal(1).DataType_internal = 'uint8'
  GroundCheckoutLink.Elements_internal(1).Complexity = 'real'
  GroundCheckoutLink.Elements_internal(1).Dimensions = 1
  GroundCheckoutLink.Elements_internal(2) = Simulink.BusElement
  GroundCheckoutLink.Elements_internal(2).DimensionsMode = 'Fixed'
  GroundCheckoutLink.Elements_internal(2).SamplingMode = 'Sample based'
  GroundCheckoutLink.Elements_internal(2).SampleTime = -1
  GroundCheckoutLink.Elements_internal(2).Description = '{Uplink, Downlink}'
  GroundCheckoutLink.Elements_internal(2).Name = 'direction'
  GroundCheckoutLink.Elements_internal(2).DataType_internal = 'enumration'
  GroundCheckoutLink.Elements_internal(2).Complexity = 'real'
  GroundCheckoutLink.Elements_internal(2).Dimensions = 1
  GroundCheckoutLink.Elements_internal(3) = Simulink.BusElement
  GroundCheckoutLink.Elements_internal(3).DimensionsMode = 'Fixed'
  GroundCheckoutLink.Elements_internal(3).SamplingMode = 'Sample based'
  GroundCheckoutLink.Elements_internal(3).SampleTime = -1
  GroundCheckoutLink.Elements_internal(3).Name = 'status'
  GroundCheckoutLink.Elements_internal(3).DataType_internal = 'uint8'
  GroundCheckoutLink.Elements_internal(3).Complexity = 'real'
  GroundCheckoutLink.Elements_internal(3).Dimensions = 1
  GroundCheckoutLink.DataScope = 'Auto'
  GroundPressurantSupply = Simulink.ConnectionBus
  GroundPressurantSupply.Elements_internal = Simulink.ConnectionElement
  GroundPressurantSupply.Elements_internal.Name = 'Element'
  GroundPressurantSupply.Elements_internal.Type_internal = 'Connection: foundation.gas.gas'
  GuidanceConstraints = Simulink.Bus
  GuidanceConstraints.Alignment = -1
  GuidanceConstraints.PreserveElementDimensions = 0
  GuidanceConstraints.Elements_internal(1) = Simulink.BusElement
  GuidanceConstraints.Elements_internal(1).DimensionsMode = 'Fixed'
  GuidanceConstraints.Elements_internal(1).SamplingMode = 'Sample based'
  GuidanceConstraints.Elements_internal(1).SampleTime = -1
  GuidanceConstraints.Elements_internal(1).Name = 'constraintID'
  GuidanceConstraints.Elements_internal(1).DataType_internal = 'uint16'
  GuidanceConstraints.Elements_internal(1).Complexity = 'real'
  GuidanceConstraints.Elements_internal(1).Dimensions = 1
  GuidanceConstraints.Elements_internal(2) = Simulink.BusElement
  GuidanceConstraints.Elements_internal(2).DimensionsMode = 'Fixed'
  GuidanceConstraints.Elements_internal(2).SamplingMode = 'Sample based'
  GuidanceConstraints.Elements_internal(2).SampleTime = -1
  GuidanceConstraints.Elements_internal(2).Name = 'limitVector'
  GuidanceConstraints.Elements_internal(2).DataType_internal = 'double'
  GuidanceConstraints.Elements_internal(2).Complexity = 'real'
  GuidanceConstraints.Elements_internal(2).Dimensions = 1
  GuidanceConstraints.Elements_internal(3) = Simulink.BusElement
  GuidanceConstraints.Elements_internal(3).DimensionsMode = 'Fixed'
  GuidanceConstraints.Elements_internal(3).SamplingMode = 'Sample based'
  GuidanceConstraints.Elements_internal(3).SampleTime = -1
  GuidanceConstraints.Elements_internal(3).Name = 'validity'
  GuidanceConstraints.Elements_internal(3).DataType_internal = 'uint8'
  GuidanceConstraints.Elements_internal(3).Complexity = 'real'
  GuidanceConstraints.Elements_internal(3).Dimensions = 1
  GuidanceConstraints.Elements_internal(4) = Simulink.BusElement
  GuidanceConstraints.Elements_internal(4).DimensionsMode = 'Fixed'
  GuidanceConstraints.Elements_internal(4).SamplingMode = 'Sample based'
  GuidanceConstraints.Elements_internal(4).SampleTime = -1
  GuidanceConstraints.Elements_internal(4).DocUnits = 's'
  GuidanceConstraints.Elements_internal(4).Name = 'timestamp'
  GuidanceConstraints.Elements_internal(4).DataType_internal = 'double'
  GuidanceConstraints.Elements_internal(4).Complexity = 'real'
  GuidanceConstraints.Elements_internal(4).Dimensions = 1
  GuidanceConstraints.DataScope = 'Auto'
  GuidanceMode = Simulink.ValueType
  GuidanceMode.DataType = 'enumration'
  LinkHealth = Simulink.Bus
  LinkHealth.Alignment = -1
  LinkHealth.PreserveElementDimensions = 0
  LinkHealth.Elements_internal(1) = Simulink.BusElement
  LinkHealth.Elements_internal(1).DimensionsMode = 'Fixed'
  LinkHealth.Elements_internal(1).SamplingMode = 'Sample based'
  LinkHealth.Elements_internal(1).SampleTime = -1
  LinkHealth.Elements_internal(1).Description = '{Relay, DirectRF}'
  LinkHealth.Elements_internal(1).Name = 'activePath'
  LinkHealth.Elements_internal(1).DataType_internal = 'enumration'
  LinkHealth.Elements_internal(1).Complexity = 'real'
  LinkHealth.Elements_internal(1).Dimensions = 1
  LinkHealth.Elements_internal(2) = Simulink.BusElement
  LinkHealth.Elements_internal(2).DimensionsMode = 'Fixed'
  LinkHealth.Elements_internal(2).SamplingMode = 'Sample based'
  LinkHealth.Elements_internal(2).SampleTime = -1
  LinkHealth.Elements_internal(2).Name = 'signalQuality'
  LinkHealth.Elements_internal(2).DataType_internal = 'double'
  LinkHealth.Elements_internal(2).Complexity = 'real'
  LinkHealth.Elements_internal(2).Dimensions = 1
  LinkHealth.Elements_internal(3) = Simulink.BusElement
  LinkHealth.Elements_internal(3).DimensionsMode = 'Fixed'
  LinkHealth.Elements_internal(3).SamplingMode = 'Sample based'
  LinkHealth.Elements_internal(3).SampleTime = -1
  LinkHealth.Elements_internal(3).DocUnits = 's'
  LinkHealth.Elements_internal(3).Name = 'lastHandoffTime'
  LinkHealth.Elements_internal(3).DataType_internal = 'double'
  LinkHealth.Elements_internal(3).Complexity = 'real'
  LinkHealth.Elements_internal(3).Dimensions = 1
  LinkHealth.Elements_internal(4) = Simulink.BusElement
  LinkHealth.Elements_internal(4).DimensionsMode = 'Fixed'
  LinkHealth.Elements_internal(4).SamplingMode = 'Sample based'
  LinkHealth.Elements_internal(4).SampleTime = -1
  LinkHealth.Elements_internal(4).Name = 'status'
  LinkHealth.Elements_internal(4).DataType_internal = 'uint8'
  LinkHealth.Elements_internal(4).Complexity = 'real'
  LinkHealth.Elements_internal(4).Dimensions = 1
  LinkHealth.DataScope = 'Auto'
  LiquidPropellantFeed : Simulink.ConnectionBus (value not decoded)
  MechanicalMotion : Simulink.ConnectionBus (value not decoded)
  MechanismPosition : Simulink.Bus (value not decoded)
  ModeTransitionContext : Simulink.Bus (value not decoded)
  NavigationAidingData : Simulink.Bus (value not decoded)
  NavigationEstimate : Simulink.Bus (value not decoded)
  NavigationHealthStatus : Simulink.Bus (value not decoded)
  NavigationMeasurementSet : Simulink.Bus (value not decoded)
  PercentThrottle = Simulink.ValueType
  PercentThrottle.Min = 0
  PercentThrottle.Max = 100
  PercentThrottle.Unit = '%'
  PneumaticActuationGas : Simulink.ConnectionBus (value not decoded)
  PowerConversionStatus : Simulink.Bus (value not decoded)
  PowerDistributionStatus : Simulink.Bus (value not decoded)
  PowerHealthStatus : Simulink.Bus (value not decoded)
  PowerManagementCommand : Simulink.Bus (value not decoded)
  PowerStorageStatus : Simulink.Bus (value not decoded)
  ProtectedThermalState : Simulink.Bus (value not decoded)
  ProtectionIsolationStatus : Simulink.Bus (value not decoded)
  PurgeGasSupply : Simulink.ConnectionBus (value not decoded)
  RCSPulseCommand : Simulink.Bus (value not decoded)
  RCSTelemetry : Simulink.Bus (value not decoded)
  RFFeed : Simulink.ConnectionBus (value not decoded)
  RecoveryMechanismCommand : Simulink.Bus (value not decoded)
  RollThrottleBias : Simulink.ValueType (value not decoded)
  SafetyOverride : Simulink.ValueType (value not decoded)
  SafetyStateStatus : Simulink.Bus (value not decoded)
  ShapedControlDemand : Simulink.Bus (value not decoded)
  SpinStartIgniterGas : Simulink.ConnectionBus (value not decoded)
  StageMechanicalBoundary : Simulink.ConnectionBus (value not decoded)
  StructuralLoad : Simulink.ConnectionBus (value not decoded)
  StructureHealthStatus : Simulink.Bus (value not decoded)
  SubsystemHealthEvidence : Simulink.Bus (value not decoded)
  SubsystemStatusTelemetry : Simulink.Bus (value not decoded)
  TankTelemetry : Simulink.Bus (value not decoded)
  ThermalMonitoringCommand : Simulink.Bus (value not decoded)
  ThermalNetwork : Simulink.ConnectionBus (value not decoded)
  ThrustLoad : Simulink.ConnectionBus (value not decoded)
  TrajectoryGuidanceCommand : Simulink.Bus (value not decoded)
  TrajectoryReference : Simulink.Bus (value not decoded)
  TranslationalControlDemand : Simulink.Bus (value not decoded)
  TranslationalState : Simulink.Bus (value not decoded)
  UplinkSignal : Simulink.Bus (value not decoded)
  ValidatedControlDemand : Simulink.Bus (value not decoded)
  ValveCommand : Simulink.ValueType (value not decoded)
  VehicleStructureState : Simulink.Bus (value not decoded)
  VerifiedCommand : Simulink.Bus (value not decoded)
  VideoStream : Simulink.Bus (value not decoded)
undefined symbols (not defined in the file): ACR, ACT, ASM, ATM, BCR, BDQ, BDR, BDX, BEC, BFC, BHV, BIP, BLM, BNZ, BPI, BPR, BPV, BRX, BSM, BTA, BTP, BVC, BVE, BVV, CAA, CAM, CAS, CAT, CLM, COM, CRS, CTL, CTR, DAQ, ESC, EXT, FCR, FDB, FDE, FEX, FHI, FHM, FIC, FIS, FMG, FSC, GAP, GCM, GMD, GNC, GND, GPH, GTR, HDN, HIA, HSI, IF, INT, LOC, NAI ... (+45)
(part 1 of 8)
settings Model: Creator=ASUS  LastModifiedBy=ASUS

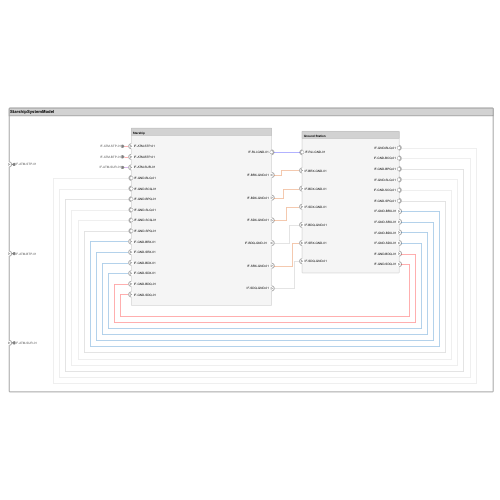
[thumbnail: Simulink's stored preview of the top-level diagram]
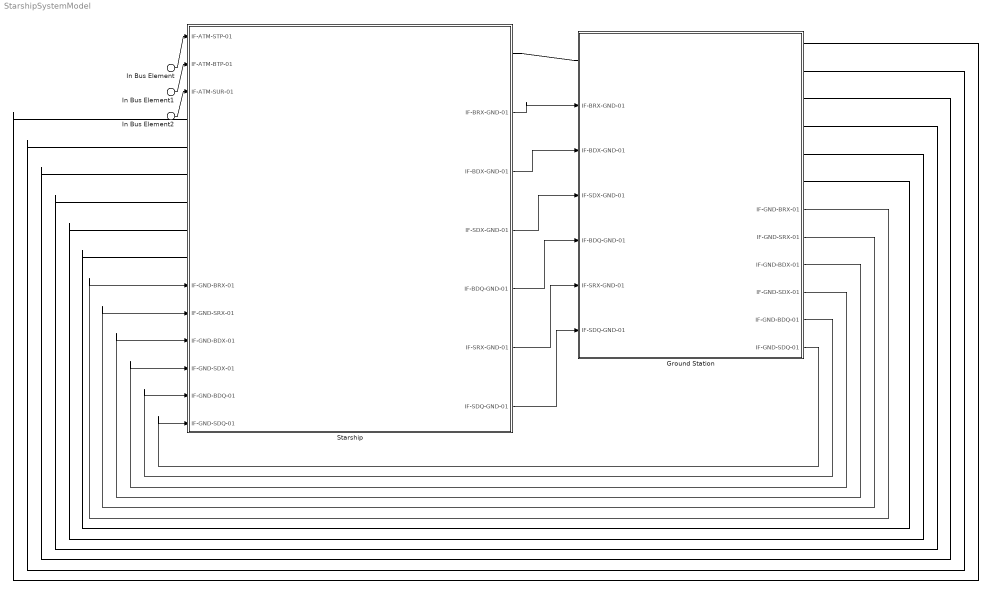
== system StarshipSystemModel ==
  In Bus Element : Inport  PortName=IF-ATM-STP-01
  In Bus Element1 : Inport  Port=2  PortName=IF-ATM-BTP-01
  In Bus Element2 : Inport  Port=3  PortName=IF-ATM-SUR-01
  Ground Station : Subsystem
      settings: PortSchema="{\"entries\":[{\"content\":{\"headerSize\":26,\"margin\":15,\"minimumSpacing\":25,\"sides\":[{\"content\":{\"connectorIds\":[\"LConn1\",\"In1\",\"In2\",\"In3\",\"In4\",\"In5\",\"In6\"]},\"type\":\"ConnectorPlacement.EquallySpacedRectSide\",\"uuid\":\"a24f90f9-b52e-4407-98a2-61cef3ed1001\"},{\"content\":{\"connectorIds\":[\"RConn1\",\"RConn2\",\"RConn3\",\"RConn4\",\"RConn5\",\"RConn6\",\"Out1\",\"Out2\",\"Out3\",\"Out4\",\"Out5\",\"Out6\"],\"side\":\"RIGHT\"},\"type\":\"ConnectorPlacement.EquallySpacedRectSide\",\"uuid\":\"349c89d4-9966-4ad9-ba76-db4d38641e72\"},{\"content\":{\"side\":\"TOP\"},\"type\":\"ConnectorPlacement.EquallySpacedRectSide\",\"uuid\":\"c23b8a3e-5693-4bb4-96b3-90d999333c4e\"}]},\"type\":\"ConnectorPlacement.EquallySpacedConnector\",\"uuid\":\"ab682651-c32f-4460-8c4f-01dcf64563ad\"}],\"packageUris\":[\"http://schema.mathworks.com/mf0/Connector/R2020b\"],\"version\":\"1.0\"}"
  Starship : Subsystem
      settings: PortSchema="{\"entries\":[{\"content\":{\"headerSize\":26,\"margin\":15,\"minimumSpacing\":25,\"sides\":[{\"content\":{\"connectorIds\":[\"In1\",\"In2\",\"In9\",\"LConn1\",\"LConn2\",\"LConn3\",\"LConn4\",\"LConn5\",\"LConn6\",\"In3\",\"In4\",\"In5\",\"In6\",\"In7\",\"In8\"]},\"type\":\"ConnectorPlacement.EquallySpacedRectSide\",\"uuid\":\"a24f90f9-b52e-4407-98a2-61cef3ed1001\"},{\"content\":{\"connectorIds\":[\"RConn1\",\"Out1\",\"Out2\",\"Out3\",\"Out4\",\"Out5\",\"Out6\"],\"side\":\"RIGHT\"},\"type\":\"ConnectorPlacement.EquallySpacedRectSide\",\"uuid\":\"349c89d4-9966-4ad9-ba76-db4d38641e72\"},{\"content\":{\"side\":\"TOP\"},\"type\":\"ConnectorPlacement.EquallySpacedRectSide\",\"uuid\":\"c23b8a3e-5693-4bb4-96b3-90d999333c4e\"}]},\"type\":\"ConnectorPlacement.EquallySpacedConnector\",\"uuid\":\"ab682651-c32f-4460-8c4f-01dcf64563ad\"}],\"packageUris\":[\"http://schema.mathworks.com/mf0/Connector/R2020b\"],\"version\":\"1.0\"}"
  wires:
  Starship/1(IF-BRX-GND-01) -> Ground Station/1(IF-BRX-GND-01)
  In Bus Element/1 -> Starship/1(IF-ATM-STP-01)
  In Bus Element1/1 -> Starship/2(IF-ATM-BTP-01)
  In Bus Element2/1 -> Starship/9(IF-ATM-SUR-01)
  Starship/6(IF-SDQ-GND-01) -> Ground Station/6(IF-SDQ-GND-01)
  Starship/2(IF-BDX-GND-01) -> Ground Station/2(IF-BDX-GND-01)
  Starship/4("IF-BDQ-GND-01\t") -> Ground Station/4("IF-BDQ-GND-01\t")
  Starship/5(IF-SRX-GND-01) -> Ground Station/5(IF-SRX-GND-01)
  Starship/3(IF-SDX-GND-01) -> Ground Station/3(IF-SDX-GND-01)
  Ground Station/5(IF-GND-BDQ-01) -> Starship/7(IF-GND-BDQ-01)
  Ground Station/3(IF-GND-BDX-01) -> Starship/5(IF-GND-BDX-01)
  Ground Station/6(IF-GND-SDQ-01) -> Starship/8(IF-GND-SDQ-01)
  Ground Station/4(IF-GND-SDX-01) -> Starship/6(IF-GND-SDX-01)
  Ground Station/1(IF-GND-BRX-01) -> Starship/3(IF-GND-BRX-01)
  Ground Station/2(IF-GND-SRX-01) -> Starship/4(IF-GND-SRX-01)
  connections:
  Starship/RConn1 -- Ground Station/LConn1
  Ground Station/RConn3 -- Starship/LConn3
  Ground Station/RConn1 -- Starship/LConn1
  Ground Station/RConn4 -- Starship/LConn4
  Ground Station/RConn2 -- Starship/LConn2
  Ground Station/RConn5 -- Starship/LConn5
  Ground Station/RConn6 -- Starship/LConn6

== system StarshipSystemModel/Ground Station ==
  Bus Element In1 : Inport  PortName=IF-BRX-GND-01
  Bus Element In3 : Inport  Port=2  PortName=IF-BDX-GND-01
  Bus Element In4 : Inport  Port=3  PortName=IF-SDX-GND-01
  Bus Element In5 : Inport  Port=4  PortName=IF-BDQ-GND-01
  Bus Element In2 : Inport  Port=5  PortName=IF-SRX-GND-01
  Bus Element In6 : Inport  Port=6  PortName=IF-SDQ-GND-01
  IF-GND-BLQ-01 : PMIOPort  Side=Right
  IF-GND-BCQ-01 : PMIOPort  Port=2  Side=Right
  IF-GND-BPQ-01 : PMIOPort  Port=3  Side=Right  ConnectionType=Bus: GroundPressurantSupply
  IF-GND-SLQ-01 : PMIOPort  Port=4  Side=Right
  IF-GND-SCQ-01 : PMIOPort  Port=5  Side=Right
  IF-GND-SPQ-01 : PMIOPort  Port=6  Side=Right  ConnectionType=Bus: GroundPressurantSupply
  IF-RLI-GND-01 : PMIOPort  Port=7  Side=Left  ConnectionType=Bus: StructuralLoad
  Bus Element Out1 : Outport  PortName=IF-GND-BRX-01
  Bus Element Out2 : Outport  Port=2  PortName=IF-GND-SRX-01
  Bus Element Out3 : Outport  Port=3  PortName=IF-GND-BDX-01
  Bus Element Out4 : Outport  Port=4  PortName=IF-GND-SDX-01
  Bus Element Out5 : Outport  Port=5  PortName=IF-GND-BDQ-01
  Bus Element Out6 : Outport  Port=6  PortName=IF-GND-SDQ-01

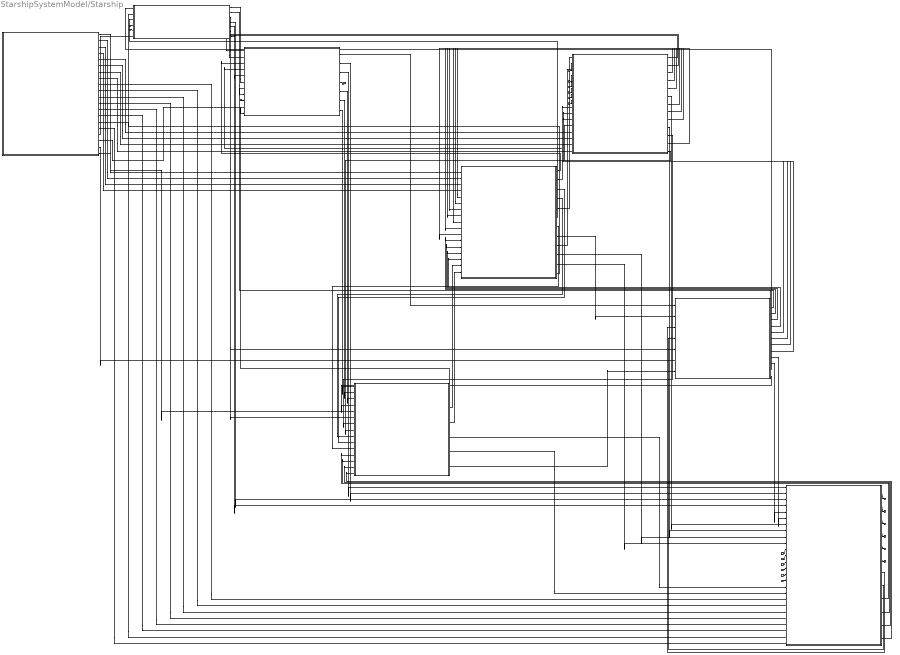
== system StarshipSystemModel/Starship ==
  Bus Element In7 : Inport  PortName=IF-ATM-STP-01
  Bus Element In8 : Inport  Port=2  PortName=IF-ATM-BTP-01
  Bus Element In1 : Inport  Port=3  PortName=IF-GND-BRX-01
  Bus Element In2 : Inport  Port=4  PortName=IF-GND-SRX-01
  Bus Element In3 : Inport  Port=5  PortName=IF-GND-BDX-01
  Bus Element In4 : Inport  Port=6  PortName=IF-GND-SDX-01
  Bus Element In5 : Inport  Port=7  PortName=IF-GND-BDQ-01
  Bus Element In6 : Inport  Port=8  PortName=IF-GND-SDQ-01
  Bus Element In9 : Inport  Port=9  PortName=IF-ATM-SUR-01
  Communications : Subsystem
      settings: PortSchema="{\"entries\":[{\"content\":{\"headerSize\":26,\"margin\":15,\"minimumSpacing\":25,\"sides\":[{\"content\":{\"connectorIds\":[\"In1\",\"In2\",\"In3\",\"In4\",\"In5\",\"In6\",\"In7\",\"In8\",\"In9\",\"In10\",\"In11\",\"In12\",\"In13\",\"In14\",\"In15\",\"In16\",\"In17\",\"In18\",\"LConn1\",\"LConn2\",\"LConn3\",\"LConn4\",\"LConn5\",\"LConn6\",\"LConn7\",\"LConn8\"]},\"type\":\"ConnectorPlacement.EquallySpacedRectSide\",\"uuid\":\"a24f90f9-b52e-4407-98a2-61cef3ed1001\"},{\"content\":{\"connectorIds\":[\"Out1\",\"Out2\",\"Out3\",\"Out4\",\"Out5\",\"Out6\",\"Out7\",\"Out8\",\"Out9\",\"Out10\",\"Out11\",\"Out12\"],\"side\":\"RIGHT\"},\"type\":\"ConnectorPlacement.EquallySpacedRectSide\",\"uuid\":\"349c89d4-9966-4ad9-ba76-db4d38641e72\"},{\"content\":{\"side\":\"TOP\"},\"type\":\"ConnectorPlacement.EquallySpacedRectSide\",\"uuid\":\"c23b8a3e-5693-4bb4-96b3-90d999333c4e\"}]},\"type\":\"ConnectorPlacement.EquallySpacedConnector\",\"uuid\":\"ab682651-c32f-4460-8c4f-01dcf64563ad\"}],\"packageUris\":[\"http://schema.mathworks.com/mf0/Connector/R2020b\"],\"version\":\"1.0\"}"
  GNC : Subsystem
      settings: PortSchema="{\"entries\":[{\"content\":{\"headerSize\":26,\"margin\":15,\"minimumSpacing\":25,\"sides\":[{\"content\":{\"connectorIds\":[\"In1\",\"In2\",\"In3\",\"In4\",\"In5\",\"LConn1\",\"In6\"]},\"type\":\"ConnectorPlacement.EquallySpacedRectSide\",\"uuid\":\"a24f90f9-b52e-4407-98a2-61cef3ed1001\"},{\"content\":{\"connectorIds\":[\"Out1\",\"Out2\",\"Out3\",\"Out4\",\"Out5\",\"Out6\",\"Out7\",\"Out8\",\"Out9\",\"Out10\",\"Out11\",\"Out12\",\"Out13\"],\"side\":\"RIGHT\"},\"type\":\"ConnectorPlacement.EquallySpacedRectSide\",\"uuid\":\"349c89d4-9966-4ad9-ba76-db4d38641e72\"},{\"content\":{\"side\":\"TOP\"},\"type\":\"ConnectorPlacement.EquallySpacedRectSide\",\"uuid\":\"c23b8a3e-5693-4bb4-96b3-90d999333c4e\"}]},\"type\":\"ConnectorPlacement.EquallySpacedConnector\",\"uuid\":\"ab682651-c32f-4460-8c4f-01dcf64563ad\"}],\"packageUris\":[\"http://schema.mathworks.com/mf0/Connector/R2020b\"],\"version\":\"1.0\"}"
  Power & Electrical Energy : Subsystem
      settings: PortSchema="{\"entries\":[{\"content\":{\"headerSize\":26,\"margin\":15,\"minimumSpacing\":25,\"sides\":[{\"content\":{},\"type\":\"ConnectorPlacement.EquallySpacedRectSide\",\"uuid\":\"a24f90f9-b52e-4407-98a2-61cef3ed1001\"},{\"content\":{\"connectorIds\":[\"RConn1\",\"RConn2\",\"RConn3\",\"RConn4\",\"RConn6\",\"RConn5\",\"RConn7\",\"RConn8\",\"RConn9\",\"RConn10\",\"RConn11\",\"RConn12\",\"RConn13\",\"RConn14\",\"RConn15\",\"RConn16\",\"RConn17\",\"RConn18\",\"RConn19\",\"Out1\"],\"side\":\"RIGHT\"},\"type\":\"ConnectorPlacement.EquallySpacedRectSide\",\"uuid\":\"349c89d4-9966-4ad9-ba76-db4d38641e72\"},{\"content\":{\"side\":\"TOP\"},\"type\":\"ConnectorPlacement.EquallySpacedRectSide\",\"uuid\":\"c23b8a3e-5693-4bb4-96b3-90d999333c4e\"}]},\"type\":\"ConnectorPlacement.EquallySpacedConnector\",\"uuid\":\"ab682651-c32f-4460-8c4f-01dcf64563ad\"}],\"packageUris\":[\"http://schema.mathworks.com/mf0/Connector/R2020b\"],\"version\":\"1.0\"}"
  Propellent system : Subsystem
      settings: PortSchema="{\"entries\":[{\"content\":{\"headerSize\":26,\"margin\":15,\"minimumSpacing\":25,\"sides\":[{\"content\":{\"connectorIds\":[\"LConn3\",\"LConn4\",\"LConn5\",\"LConn6\",\"LConn7\",\"LConn8\",\"LConn13\",\"LConn14\",\"In1\",\"In2\",\"In3\",\"In4\",\"LConn9\",\"LConn10\",\"LConn11\",\"LConn12\"]},\"type\":\"ConnectorPlacement.EquallySpacedRectSide\",\"uuid\":\"a24f90f9-b52e-4407-98a2-61cef3ed1001\"},{\"content\":{\"connectorIds\":[\"LConn2\",\"LConn1\",\"RConn1\",\"RConn4\",\"RConn3\",\"Out1\",\"RConn5\",\"RConn2\",\"RConn7\",\"Out2\",\"Out3\",\"RConn6\",\"Out4\"],\"side\":\"RIGHT\"},\"type\":\"ConnectorPlacement.EquallySpacedRectSide\",\"uuid\":\"349c89d4-9966-4ad9-ba76-db4d38641e72\"},{\"content\":{\"side\":\"TOP\"},\"type\":\"ConnectorPlacement.EquallySpacedRectSide\",\"uuid\":\"c23b8a3e-5693-4bb4-96b3-90d999333c4e\"}]},\"type\":\"ConnectorPlacement.EquallySpacedConnector\",\"uuid\":\"ab682651-c32f-4460-8c4f-01dcf64563ad\"}],\"packageUris\":[\"http://schema.mathworks.com/mf0/Connector/R2020b\"],\"version\":\"1.0\"}"
  Propulsion : Subsystem
      settings: PortSchema="{\"entries\":[{\"content\":{\"headerSize\":26,\"margin\":15,\"minimumSpacing\":25,\"sides\":[{\"content\":{\"connectorIds\":[\"LConn1\",\"LConn2\",\"LConn3\",\"LConn4\",\"LConn7\",\"LConn8\",\"LConn9\",\"LConn10\",\"LConn11\",\"LConn12\",\"LConn13\",\"In1\",\"In2\",\"In3\",\"In4\",\"In5\",\"In6\"]},\"type\":\"ConnectorPlacement.EquallySpacedRectSide\",\"uuid\":\"a24f90f9-b52e-4407-98a2-61cef3ed1001\"},{\"content\":{\"connectorIds\":[\"LConn6\",\"LConn5\",\"Out1\",\"Out4\",\"RConn1\",\"Out3\",\"Out7\",\"Out5\",\"RConn2\",\"Out6\",\"Out2\",\"Out8\"],\"side\":\"RIGHT\"},\"type\":\"ConnectorPlacement.EquallySpacedRectSide\",\"uuid\":\"349c89d4-9966-4ad9-ba76-db4d38641e72\"},{\"content\":{\"side\":\"TOP\"},\"type\":\"ConnectorPlacement.EquallySpacedRectSide\",\"uuid\":\"c23b8a3e-5693-4bb4-96b3-90d999333c4e\"}]},\"type\":\"ConnectorPlacement.EquallySpacedConnector\",\"uuid\":\"ab682651-c32f-4460-8c4f-01dcf64563ad\"}],\"packageUris\":[\"http://schema.mathworks.com/mf0/Connector/R2020b\"],\"version\":\"1.0\"}"
  "Safety & Fault Management " : Subsystem
      settings: PortSchema="{\"entries\":[{\"content\":{\"headerSize\":26,\"margin\":15,\"minimumSpacing\":25,\"sides\":[{\"content\":{\"connectorIds\":[\"In1\",\"In2\",\"In3\",\"In4\",\"In5\",\"In6\",\"In7\",\"In8\",\"In9\",\"In10\",\"In11\",\"In12\",\"In13\",\"In14\",\"In15\"]},\"type\":\"ConnectorPlacement.EquallySpacedRectSide\",\"uuid\":\"a24f90f9-b52e-4407-98a2-61cef3ed1001\"},{\"content\":{\"connectorIds\":[\"Out1\",\"Out4\",\"Out2\",\"Out3\",\"Out5\",\"Out6\"],\"side\":\"RIGHT\"},\"type\":\"ConnectorPlacement.EquallySpacedRectSide\",\"uuid\":\"349c89d4-9966-4ad9-ba76-db4d38641e72\"},{\"content\":{\"side\":\"TOP\"},\"type\":\"ConnectorPlacement.EquallySpacedRectSide\",\"uuid\":\"c23b8a3e-5693-4bb4-96b3-90d999333c4e\"}]},\"type\":\"ConnectorPlacement.EquallySpacedConnector\",\"uuid\":\"ab682651-c32f-4460-8c4f-01dcf64563ad\"}],\"packageUris\":[\"http://schema.mathworks.com/mf0/Connector/R2020b\"],\"version\":\"1.0\"}"
  Structure and Mechanisms : Subsystem
      settings: PortSchema="{\"entries\":[{\"content\":{\"headerSize\":26,\"margin\":15,\"minimumSpacing\":25,\"sides\":[{\"content\":{\"connectorIds\":[\"RConn4\",\"RConn3\",\"RConn2\",\"RConn1\",\"LConn1\",\"LConn2\",\"LConn3\",\"In1\",\"In2\",\"LConn4\",\"In3\"]},\"type\":\"ConnectorPlacement.EquallySpacedRectSide\",\"uuid\":\"a24f90f9-b52e-4407-98a2-61cef3ed1001\"},{\"content\":{\"connectorIds\":[\"Out1\",\"Out2\",\"Out3\",\"RConn5\",\"Out4\",\"Out5\",\"Out6\"],\"side\":\"RIGHT\"},\"type\":\"ConnectorPlacement.EquallySpacedRectSide\",\"uuid\":\"349c89d4-9966-4ad9-ba76-db4d38641e72\"},{\"content\":{\"side\":\"TOP\"},\"type\":\"ConnectorPlacement.EquallySpacedRectSide\",\"uuid\":\"c23b8a3e-5693-4bb4-96b3-90d999333c4e\"}]},\"type\":\"ConnectorPlacement.EquallySpacedConnector\",\"uuid\":\"ab682651-c32f-4460-8c4f-01dcf64563ad\"}],\"packageUris\":[\"http://schema.mathworks.com/mf0/Connector/R2020b\"],\"version\":\"1.0\"}"
  Thermal Protection : Subsystem
      settings: PortSchema="{\"entries\":[{\"content\":{\"headerSize\":26,\"margin\":15,\"minimumSpacing\":25,\"sides\":[{\"content\":{\"connectorIds\":[\"In1\",\"In2\",\"In3\",\"In4\",\"In5\",\"LConn1\"]},\"type\":\"ConnectorPlacement.EquallySpacedRectSide\",\"uuid\":\"a24f90f9-b52e-4407-98a2-61cef3ed1001\"},{\"content\":{\"connectorIds\":[\"RConn1\",\"RConn2\",\"Out1\",\"Out2\",\"Out3\",\"Out4\",\"RConn3\"],\"side\":\"RIGHT\"},\"type\":\"ConnectorPlacement.EquallySpacedRectSide\",\"uuid\":\"349c89d4-9966-4ad9-ba76-db4d38641e72\"},{\"content\":{\"side\":\"TOP\"},\"type\":\"ConnectorPlacement.EquallySpacedRectSide\",\"uuid\":\"c23b8a3e-5693-4bb4-96b3-90d999333c4e\"}]},\"type\":\"ConnectorPlacement.EquallySpacedConnector\",\"uuid\":\"ab682651-c32f-4460-8c4f-01dcf64563ad\"}],\"packageUris\":[\"http://schema.mathworks.com/mf0/Connector/R2020b\"],\"version\":\"1.0\"}"
  IF-GND-BLQ-01 : PMIOPort  Side=Left
  IF-GND-BCQ-01 : PMIOPort  Port=2  Side=Left
  IF-GND-BPQ-01 : PMIOPort  Port=3  Side=Left  ConnectionType=Bus: GroundPressurantSupply
  IF-GND-SLQ-01 : PMIOPort  Port=4  Side=Left
  IF-GND-SCQ-01 : PMIOPort  Port=5  Side=Left
  IF-GND-SPQ-01 : PMIOPort  Port=6  Side=Left  ConnectionType=Bus: GroundPressurantSupply
  IF-RLI-GND-01 : PMIOPort  Port=7  Side=Right  ConnectionType=Bus: StructuralLoad
  Bus Element Out2 : Outport  PortName=IF-BRX-GND-01
  Bus Element Out3 : Outport  Port=2  PortName=IF-BDX-GND-01
  Bus Element Out4 : Outport  Port=3  PortName=IF-SDX-GND-01
  Bus Element Out5 : Outport  Port=4  PortName=IF-BDQ-GND-01
  Bus Element Out1 : Outport  Port=5  PortName=IF-SRX-GND-01
  Bus Element Out6 : Outport  Port=6  PortName=IF-SDQ-GND-01
  wires:
  Propulsion/1(IF-RCT-SAF-01) -> "Safety & Fault Management "/10(IF-RCT-SAF-01)
  Bus Element In7/1 -> Thermal Protection/4(IF-ATM-STP-01)
  Bus Element In8/1 -> Thermal Protection/5(IF-ATM-BTP-01)
  Propulsion/4(IF-BEC-SAF-01) -> "Safety & Fault Management "/9(IF-BEC-SAF-01)
  Propulsion/2(IF-BEC-BTA-01) -> Communications/10(IF-BEC-BTA-01)
  GNC/5(IF-GNC-RCT-01) -> Propulsion/4(IF-GNC-RCT-01)
  Propulsion/6(IF-SEC-STA-01) -> Communications/9(IF-SEC-STA-01)
  Structure and Mechanisms/2(IF-INT-STA-01) -> Communications/2(IF-INT-STA-01)
  Communications/9(IF-BCR-SAF-01) -> "Safety & Fault Management "/12(IF-BCR-SAF-01)
  "Safety & Fault Management "/2(IF-SAF-SEC-01) -> Propulsion/6(IF-SAF-SEC-01)
  GNC/8(IF-GNC-BPR-01) -> Propellent system/3(IF-GNC-BPR-01)
  Propulsion/8(IF-SNZ-STP-01) -> Thermal Protection/2(IF-SNZ-STP-01)
  "Safety & Fault Management "/4(IF-SAF-BEC-01) -> Propulsion/5(IF-SAF-BEC-01)
  Power & Electrical Energy/1(IF-PMM-SAF-01) -> "Safety & Fault Management "/5(IF-PMM-SAF-01)
  Thermal Protection/1(IF-TMS-GNC-01) -> GNC/5(IF-TMS-GNC-01)
  Bus Element In9/1 -> Structure and Mechanisms/2(IF-ATM-SUR-01)
  Thermal Protection/2(IF-TMS-BTA-01) -> Communications/3(IF-TMS-BTA-01)
  Thermal Protection/3(IF-TMS-STA-01) -> Communications/4(IF-TMS-STA-01)
  Communications/10(IF-SCR-SAF-01) -> "Safety & Fault Management "/13(IF-SCR-SAF-01)
  Thermal Protection/4(IF-TMS-SAF-01) -> "Safety & Fault Management "/6(IF-TMS-SAF-01)
  "Safety & Fault Management "/5(IF-SAF-STA-01) -> Communications/18(IF-SAF-STA-01)
  Structure and Mechanisms/1(IF-POS-GNC-01) -> GNC/1(IF-POS-GNC-01)
  Structure and Mechanisms/3(IF-INT-BTA-01) -> Communications/1(IF-INT-BTA-01)
  Structure and Mechanisms/4(IF-POS-SAF-01) -> "Safety & Fault Management "/3(IF-POS-SAF-01)
  Propulsion/7(IF-SEC-SAF-01) -> "Safety & Fault Management "/11(IF-SEC-SAF-01)
  Structure and Mechanisms/5(IF-INT-SAF-01) -> "Safety & Fault Management "/2(IF-INT-SAF-01)
  Structure and Mechanisms/6(IF-RSM-SAF-01) -> "Safety & Fault Management "/1(IF-RSM-SAF-01)
  "Safety & Fault Management "/1(IF-SAF-RSM-01) -> Structure and Mechanisms/3(IF-SAF-RSM-01)
  "Safety & Fault Management "/3(IF-SAF-BTA-01) -> Communications/17(IF-SAF-BTA-01)
  "Safety & Fault Management "/6(IF-SAF-FHM-01) -> GNC/6(IF-SAF-FHM-01)
  Propellent system/1(IF-BPR-BTA-01) -> Communications/7(IF-BPR-BTA-01)
  Propulsion/3(IF-BNZ-BTP-01) -> Thermal Protection/3(IF-BNZ-BTP-01)
  Propulsion/5(IF-TVC-GNC-01) -> GNC/2(IF-TVC-GNC-01)
  Propellent system/2(IF-SPR-STA-01) -> Communications/8(IF-SPR-STA-01)
  Propellent system/3(IF-SPR-SAF-01) -> "Safety & Fault Management "/7(IF-SPR-SAF-01)
  Propellent system/4(IF-BPR-SAF-01) -> "Safety & Fault Management "/8(IF-BPR-SAF-01)
  GNC/1(IF-GNC-ACT-01) -> Structure and Mechanisms/1(IF-GNC-ACT-01)
  GNC/2(IF-GNC-BEC-01) -> Propulsion/1(IF-GNC-BEC-01)
  GNC/3(IF-GNC-SEC-01) -> Propulsion/2(IF-GNC-SEC-01)
  GNC/4(IF-GNC-TVC-01) -> Propulsion/3(IF-GNC-TVC-01)
  GNC/6(IF-GNC-BFC-01) -> Propellent system/1(IF-GNC-BFC-01)
  GNC/7(IF-GNC-SFC-01) -> Propellent system/2(IF-GNC-SFC-01)
  GNC/9(IF-GNC-SPR-01) -> Propellent system/4(IF-GNC-SPR-01)
  GNC/10(IF-GNC-BTA-01) -> Communications/6(IF-GNC-BTA-01)
  GNC/11(IF-GNC-STA-01) -> Communications/5(IF-GNC-STA-01)
  GNC/12(IF-GNC-TMS-01) -> Thermal Protection/1(IF-GNC-TMS-01)
  GNC/13(IF-FHM-SAF-01) -> "Safety & Fault Management "/4(IF-FHM-SAF-01)
  Bus Element In1/1 -> Communications/11(IF-GND-BRX-01)
  Bus Element In2/1 -> Communications/12(IF-GND-SRX-01)
  Bus Element In3/1 -> Communications/13(IF-GND-BDX-01)
  Bus Element In4/1 -> Communications/14(IF-GND-SDX-01)
  Bus Element In5/1 -> Communications/15(IF-GND-BDQ-01)
  Bus Element In6/1 -> Communications/16(IF-GND-SDQ-01)
  Communications/1(IF-BDX-GND-01) -> Bus Element Out3/1
  Communications/2(IF-BDQ-GND-01) -> Bus Element Out5/1
  Communications/3(IF-BRX-GND-01) -> Bus Element Out2/1
  Communications/4(IF-SDX-GND-01) -> Bus Element Out4/1
  Communications/5(IF-SRX-GND-01) -> Bus Element Out1/1
  Communications/6(IF-SDQ-GND-01) -> Bus Element Out6/1
  Communications/7(IF-BCR-GNC-01) -> GNC/3(IF-BCR-GNC-01)
  Communications/8(IF-SCR-GNC-01) -> GNC/4(IF-SCR-GNC-01)
  Communications/11(IF-BLM-SAF-01) -> "Safety & Fault Management "/14(IF-BLM-SAF-01)
  Communications/12(IF-SLM-SAF-01) -> "Safety & Fault Management "/15(IF-SLM-SAF-01)
  connections:
  Propellent system/LConn1 -- Structure and Mechanisms/RConn4
  Propellent system/RConn3 -- Propulsion/LConn11
  IF-GND-SPQ-01/RConn1 -- Propellent system/LConn14
  Power & Electrical Energy/RConn5 -- Propellent system/LConn10
  Power & Electrical Energy/RConn19 -- GNC/LConn1
  Power & Electrical Energy/RConn3 -- Propulsion/LConn3
  Power & Electrical Energy/RConn9 -- Communications/LConn1
  Power & Electrical Energy/RConn1 -- Propulsion/LConn1
  Propulsion/LConn6 -- Structure and Mechanisms/RConn2
  Power & Electrical Energy/RConn6 -- Propellent system/LConn9
  Power & Electrical Energy/RConn4 -- Propulsion/LConn4
  Power & Electrical Energy/RConn18 -- Structure and Mechanisms/LConn4
  Power & Electrical Energy/RConn2 -- Propulsion/LConn2
  Power & Electrical Energy/RConn7 -- Propellent system/LConn11
  IF-GND-SLQ-01/RConn1 -- Propellent system/LConn8
  Power & Electrical Energy/RConn8 -- Propellent system/LConn12
  Propulsion/RConn1 -- Propellent system/LConn3
  Power & Electrical Energy/RConn10 -- Communications/LConn2
  IF-GND-BCQ-01/RConn1 -- Propellent system/LConn6
  Power & Electrical Energy/RConn11 -- Communications/LConn3
  Power & Electrical Energy/RConn12 -- Communications/LConn4
  Power & Electrical Energy/RConn13 -- Communications/LConn5
  Power & Electrical Energy/RConn14 -- Communications/LConn6
  Power & Electrical Energy/RConn15 -- Communications/LConn7
  Structure and Mechanisms/RConn5 -- IF-RLI-GND-01/RConn1
  Power & Electrical Energy/RConn16 -- Communications/LConn8
  Power & Electrical Energy/RConn17 -- Thermal Protection/LConn1
  Thermal Protection/RConn1 -- Structure and Mechanisms/LConn2
  Thermal Protection/RConn2 -- Structure and Mechanisms/LConn3
  Thermal Protection/RConn3 -- Structure and Mechanisms/LConn1
  Propellent system/LConn2 -- Structure and Mechanisms/RConn3
  Propellent system/RConn4 -- Propulsion/LConn8
  IF-GND-BPQ-01/RConn1 -- Propellent system/LConn7
  IF-GND-BLQ-01/RConn1 -- Propellent system/LConn4
  IF-GND-SCQ-01/RConn1 -- Propellent system/LConn13
  Propulsion/LConn5 -- Structure and Mechanisms/RConn1
  Propellent system/RConn1 -- Propulsion/LConn7
  Propulsion/RConn2 -- Propellent system/LConn5
  Propellent system/RConn5 -- Propulsion/LConn9
  Propellent system/RConn2 -- Propulsion/LConn10
  Propellent system/RConn7 -- Propulsion/LConn12
  Propellent system/RConn6 -- Propulsion/LConn13

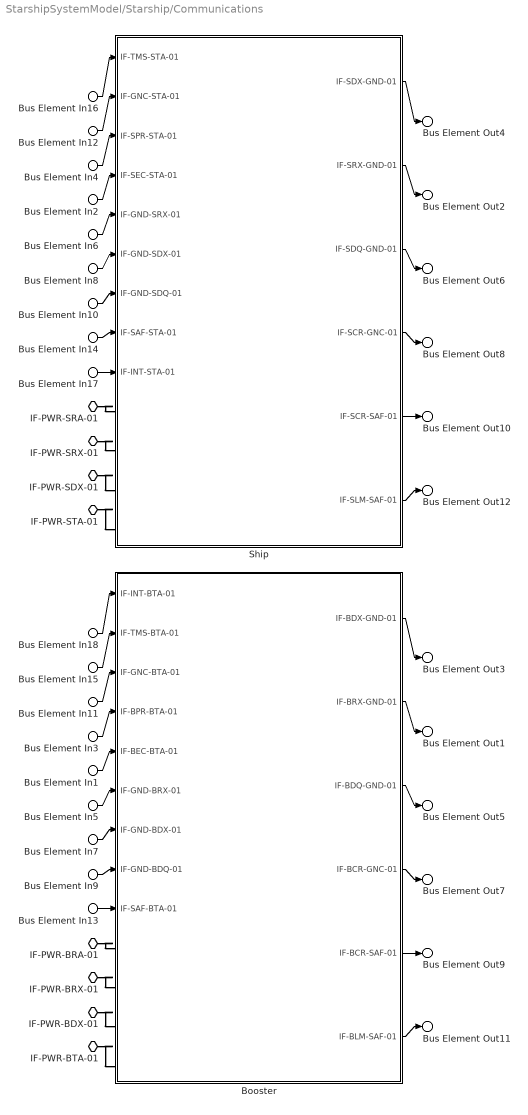
== system StarshipSystemModel/Starship/Communications ==
  Bus Element In18 : Inport  PortName=IF-INT-BTA-01
  Bus Element In17 : Inport  Port=2  PortName=IF-INT-STA-01
  Bus Element In15 : Inport  Port=3  PortName=IF-TMS-BTA-01
  Bus Element In16 : Inport  Port=4  PortName=IF-TMS-STA-01
  Bus Element In12 : Inport  Port=5  PortName=IF-GNC-STA-01
  Bus Element In11 : Inport  Port=6  PortName=IF-GNC-BTA-01
  Bus Element In3 : Inport  Port=7  PortName=IF-BPR-BTA-01
  Bus Element In4 : Inport  Port=8  PortName=IF-SPR-STA-01
  Bus Element In2 : Inport  Port=9  PortName=IF-SEC-STA-01
  Bus Element In1 : Inport  Port=10  PortName=IF-BEC-BTA-01
  Bus Element In5 : Inport  Port=11  PortName=IF-GND-BRX-01
  Bus Element In6 : Inport  Port=12  PortName=IF-GND-SRX-01
  Bus Element In7 : Inport  Port=13  PortName=IF-GND-BDX-01
  Bus Element In8 : Inport  Port=14  PortName=IF-GND-SDX-01
  Bus Element In9 : Inport  Port=15  PortName=IF-GND-BDQ-01
  Bus Element In10 : Inport  Port=16  PortName=IF-GND-SDQ-01
  Bus Element In13 : Inport  Port=17  PortName=IF-SAF-BTA-01
  Bus Element In14 : Inport  Port=18  PortName=IF-SAF-STA-01
  Booster : Subsystem
      settings: PortSchema="{\"entries\":[{\"content\":{\"headerSize\":26,\"margin\":15,\"minimumSpacing\":25,\"sides\":[{\"content\":{\"connectorIds\":[\"In1\",\"In2\",\"In3\",\"In4\",\"In5\",\"In6\",\"In7\",\"In8\",\"In9\",\"LConn1\",\"LConn2\",\"LConn3\",\"LConn4\"]},\"type\":\"ConnectorPlacement.EquallySpacedRectSide\",\"uuid\":\"57d8a002-ec9a-4125-b797-7e7c6712bf02\"},{\"content\":{\"connectorIds\":[\"Out1\",\"Out2\",\"Out3\",\"Out4\",\"Out5\",\"Out6\"],\"side\":\"RIGHT\"},\"type\":\"ConnectorPlacement.EquallySpacedRectSide\",\"uuid\":\"9c166a96-12fc-4382-8ebe-da88da7fda26\"},{\"content\":{\"side\":\"TOP\"},\"type\":\"ConnectorPlacement.EquallySpacedRectSide\",\"uuid\":\"d709cb41-f5aa-4a2a-ad2b-35894222a9c1\"}]},\"type\":\"ConnectorPlacement.EquallySpacedConnector\",\"uuid\":\"04bb3772-118b-42d1-ac15-43c1b901053a\"}],\"packageUris\":[\"http://schema.mathworks.com/mf0/Connector/R2020b\"],\"version\":\"1.0\"}"
  Ship : Subsystem
      settings: PortSchema="{\"entries\":[{\"content\":{\"headerSize\":26,\"margin\":15,\"minimumSpacing\":25,\"sides\":[{\"content\":{\"connectorIds\":[\"In1\",\"In2\",\"In3\",\"In4\",\"In5\",\"In6\",\"In7\",\"In8\",\"In9\",\"LConn1\",\"LConn2\",\"LConn3\",\"LConn4\"]},\"type\":\"ConnectorPlacement.EquallySpacedRectSide\",\"uuid\":\"57d8a002-ec9a-4125-b797-7e7c6712bf02\"},{\"content\":{\"connectorIds\":[\"Out1\",\"Out2\",\"Out3\",\"Out4\",\"Out5\",\"Out6\"],\"side\":\"RIGHT\"},\"type\":\"ConnectorPlacement.EquallySpacedRectSide\",\"uuid\":\"9c166a96-12fc-4382-8ebe-da88da7fda26\"},{\"content\":{\"side\":\"TOP\"},\"type\":\"ConnectorPlacement.EquallySpacedRectSide\",\"uuid\":\"d709cb41-f5aa-4a2a-ad2b-35894222a9c1\"}]},\"type\":\"ConnectorPlacement.EquallySpacedConnector\",\"uuid\":\"04bb3772-118b-42d1-ac15-43c1b901053a\"}],\"packageUris\":[\"http://schema.mathworks.com/mf0/Connector/R2020b\"],\"version\":\"1.0\"}"
  IF-PWR-BRA-01 : PMIOPort  Side=Left  ConnectionType=Bus: ElectricalPower
  IF-PWR-SRA-01 : PMIOPort  Port=2  Side=Left  ConnectionType=Bus: ElectricalPower
  IF-PWR-BRX-01 : PMIOPort  Port=3  Side=Left  ConnectionType=Bus: ElectricalPower
  IF-PWR-SRX-01 : PMIOPort  Port=4  Side=Left  ConnectionType=Bus: ElectricalPower
  IF-PWR-BDX-01 : PMIOPort  Port=5  Side=Left  ConnectionType=Bus: ElectricalPower
  IF-PWR-SDX-01 : PMIOPort  Port=6  Side=Left  ConnectionType=Bus: ElectricalPower
  IF-PWR-BTA-01 : PMIOPort  Port=7  Side=Left  ConnectionType=Bus: ElectricalPower
  IF-PWR-STA-01 : PMIOPort  Port=8  Side=Left  ConnectionType=Bus: ElectricalPower
  Bus Element Out3 : Outport  PortName=IF-BDX-GND-01
  Bus Element Out5 : Outport  Port=2  PortName=IF-BDQ-GND-01
  Bus Element Out1 : Outport  Port=3  PortName=IF-BRX-GND-01
  Bus Element Out4 : Outport  Port=4  PortName=IF-SDX-GND-01
  Bus Element Out2 : Outport  Port=5  PortName=IF-SRX-GND-01
  Bus Element Out6 : Outport  Port=6  PortName=IF-SDQ-GND-01
  Bus Element Out7 : Outport  Port=7  PortName=IF-BCR-GNC-01
  Bus Element Out8 : Outport  Port=8  PortName=IF-SCR-GNC-01
  Bus Element Out9 : Outport  Port=9  PortName=IF-BCR-SAF-01
  Bus Element Out10 : Outport  Port=10  PortName=IF-SCR-SAF-01
  Bus Element Out11 : Outport  Port=11  PortName=IF-BLM-SAF-01
  Bus Element Out12 : Outport  Port=12  PortName=IF-SLM-SAF-01
  wires:
  Bus Element In3/1 -> Booster/4(IF-BPR-BTA-01)
  Bus Element In15/1 -> Booster/2(IF-TMS-BTA-01)
  Bus Element In12/1 -> Ship/2(IF-GNC-STA-01)
  Bus Element In11/1 -> Booster/3(IF-GNC-BTA-01)
  Bus Element In16/1 -> Ship/1(IF-TMS-STA-01)
  Bus Element In1/1 -> Booster/5(IF-BEC-BTA-01)
  Bus Element In4/1 -> Ship/3(IF-SPR-STA-01)
  Bus Element In6/1 -> Ship/5(IF-GND-SRX-01)
  Bus Element In8/1 -> Ship/6(IF-GND-SDX-01)
  Bus Element In9/1 -> Booster/8(IF-GND-BDQ-01)
  Bus Element In7/1 -> Booster/7(IF-GND-BDX-01)
  Bus Element In5/1 -> Booster/6(IF-GND-BRX-01)
  Bus Element In2/1 -> Ship/4(IF-SEC-STA-01)
  Bus Element In14/1 -> Ship/8(IF-SAF-STA-01)
  Bus Element In10/1 -> Ship/7(IF-GND-SDQ-01)
  Bus Element In13/1 -> Booster/9(IF-SAF-BTA-01)
  Booster/6(IF-BLM-SAF-01) -> Bus Element Out11/1
  Booster/2(IF-BRX-GND-01) -> Bus Element Out1/1
  Ship/1(IF-SDX-GND-01) -> Bus Element Out4/1
  Ship/2(IF-SRX-GND-01) -> Bus Element Out2/1
  Booster/5(IF-BCR-SAF-01) -> Bus Element Out9/1
  Booster/1(IF-BDX-GND-01) -> Bus Element Out3/1
  Ship/3(IF-SDQ-GND-01) -> Bus Element Out6/1
  Ship/4(IF-SCR-GNC-01) -> Bus Element Out8/1
  Booster/4(IF-BCR-GNC-01) -> Bus Element Out7/1
  Ship/5(IF-SCR-SAF-01) -> Bus Element Out10/1
  Ship/6(IF-SLM-SAF-01) -> Bus Element Out12/1
  Booster/3(IF-BDQ-GND-01) -> Bus Element Out5/1
  Bus Element In17/1 -> Ship/9(IF-INT-STA-01)
  Bus Element In18/1 -> Booster/1(IF-INT-BTA-01)
  connections:
  IF-PWR-BRA-01/RConn1 -- Booster/LConn1
  IF-PWR-SRA-01/RConn1 -- Ship/LConn1
  IF-PWR-BRX-01/RConn1 -- Booster/LConn2
  IF-PWR-SRX-01/RConn1 -- Ship/LConn2
  IF-PWR-BDX-01/RConn1 -- Booster/LConn3
  IF-PWR-SDX-01/RConn1 -- Ship/LConn3
  IF-PWR-BTA-01/RConn1 -- Booster/LConn4
  IF-PWR-STA-01/RConn1 -- Ship/LConn4

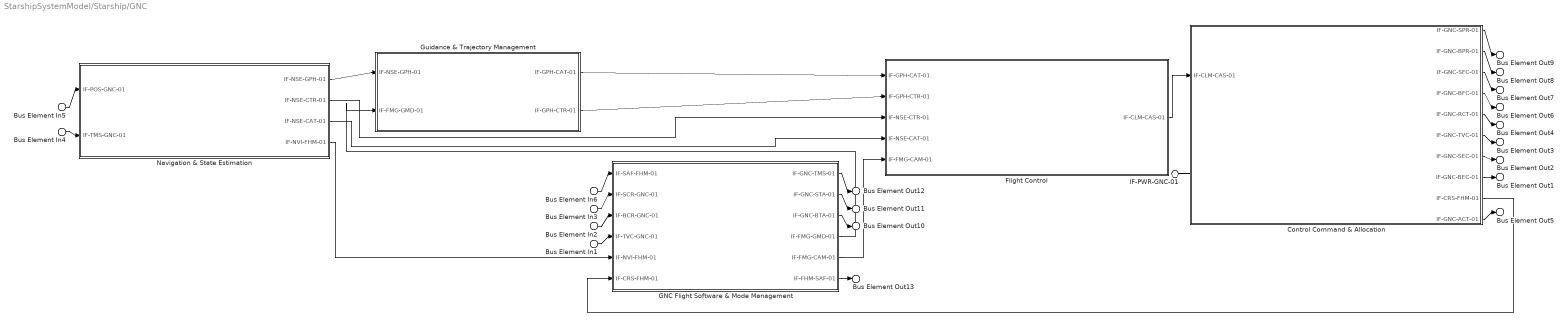
== system StarshipSystemModel/Starship/GNC ==
  Bus Element In5 : Inport  PortName=IF-POS-GNC-01
  Bus Element In1 : Inport  Port=2  PortName=IF-TVC-GNC-01
  Bus Element In2 : Inport  Port=3  PortName=IF-BCR-GNC-01
  Bus Element In3 : Inport  Port=4  PortName=IF-SCR-GNC-01
  Bus Element In4 : Inport  Port=5  PortName=IF-TMS-GNC-01
  Bus Element In6 : Inport  Port=6  PortName=IF-SAF-FHM-01
  Control Command & Allocation : Subsystem
      settings: PortSchema="{\"entries\":[{\"content\":{\"headerSize\":26,\"margin\":15,\"minimumSpacing\":25,\"sides\":[{\"content\":{\"connectorIds\":[\"In1\",\"LConn1\"]},\"type\":\"ConnectorPlacement.EquallySpacedRectSide\",\"uuid\":\"bfc9b5ca-65d3-4883-965c-09cadc06ae86\"},{\"content\":{\"connectorIds\":[\"Out1\",\"Out2\",\"Out3\",\"Out4\",\"Out5\",\"Out6\",\"Out7\",\"Out8\",\"Out9\",\"Out10\"],\"side\":\"RIGHT\"},\"type\":\"ConnectorPlacement.EquallySpacedRectSide\",\"uuid\":\"302eddba-73e5-4bab-ba05-7a4cd66d036f\"},{\"content\":{\"side\":\"TOP\"},\"type\":\"ConnectorPlacement.EquallySpacedRectSide\",\"uuid\":\"ad98d540-1dfa-45ea-9ded-5f35e32eb634\"}]},\"type\":\"ConnectorPlacement.EquallySpacedConnector\",\"uuid\":\"1bda90bf-7ec8-4676-b4c1-6df6810f307f\"}],\"packageUris\":[\"http://schema.mathworks.com/mf0/Connector/R2020b\"],\"version\":\"1.0\"}"
  Flight Control : Subsystem
      settings: PortSchema="{\"entries\":[{\"content\":{\"headerSize\":26,\"margin\":15,\"minimumSpacing\":25,\"sides\":[{\"content\":{\"connectorIds\":[\"In1\",\"In2\",\"In3\",\"In4\",\"In5\"]},\"type\":\"ConnectorPlacement.EquallySpacedRectSide\",\"uuid\":\"bfc9b5ca-65d3-4883-965c-09cadc06ae86\"},{\"content\":{\"connectorIds\":[\"Out1\"],\"side\":\"RIGHT\"},\"type\":\"ConnectorPlacement.EquallySpacedRectSide\",\"uuid\":\"302eddba-73e5-4bab-ba05-7a4cd66d036f\"},{\"content\":{\"side\":\"TOP\"},\"type\":\"ConnectorPlacement.EquallySpacedRectSide\",\"uuid\":\"ad98d540-1dfa-45ea-9ded-5f35e32eb634\"}]},\"type\":\"ConnectorPlacement.EquallySpacedConnector\",\"uuid\":\"1bda90bf-7ec8-4676-b4c1-6df6810f307f\"}],\"packageUris\":[\"http://schema.mathworks.com/mf0/Connector/R2020b\"],\"version\":\"1.0\"}"
  GNC Flight Software & Mode Management : Subsystem
      settings: PortSchema="{\"entries\":[{\"content\":{\"headerSize\":26,\"margin\":15,\"minimumSpacing\":25,\"sides\":[{\"content\":{\"connectorIds\":[\"In1\",\"In2\",\"In3\",\"In4\",\"In5\",\"In6\"]},\"type\":\"ConnectorPlacement.EquallySpacedRectSide\",\"uuid\":\"bfc9b5ca-65d3-4883-965c-09cadc06ae86\"},{\"content\":{\"connectorIds\":[\"Out1\",\"Out2\",\"Out3\",\"Out4\",\"Out5\",\"Out6\"],\"side\":\"RIGHT\"},\"type\":\"ConnectorPlacement.EquallySpacedRectSide\",\"uuid\":\"302eddba-73e5-4bab-ba05-7a4cd66d036f\"},{\"content\":{\"side\":\"TOP\"},\"type\":\"ConnectorPlacement.EquallySpacedRectSide\",\"uuid\":\"ad98d540-1dfa-45ea-9ded-5f35e32eb634\"}]},\"type\":\"ConnectorPlacement.EquallySpacedConnector\",\"uuid\":\"1bda90bf-7ec8-4676-b4c1-6df6810f307f\"}],\"packageUris\":[\"http://schema.mathworks.com/mf0/Connector/R2020b\"],\"version\":\"1.0\"}"
  Guidance & Trajectory Management : Subsystem
      settings: PortSchema="{\"entries\":[{\"content\":{\"headerSize\":26,\"margin\":15,\"minimumSpacing\":25,\"sides\":[{\"content\":{\"connectorIds\":[\"In1\",\"In2\"]},\"type\":\"ConnectorPlacement.EquallySpacedRectSide\",\"uuid\":\"bfc9b5ca-65d3-4883-965c-09cadc06ae86\"},{\"content\":{\"connectorIds\":[\"Out1\",\"Out2\"],\"side\":\"RIGHT\"},\"type\":\"ConnectorPlacement.EquallySpacedRectSide\",\"uuid\":\"302eddba-73e5-4bab-ba05-7a4cd66d036f\"},{\"content\":{\"side\":\"TOP\"},\"type\":\"ConnectorPlacement.EquallySpacedRectSide\",\"uuid\":\"ad98d540-1dfa-45ea-9ded-5f35e32eb634\"}]},\"type\":\"ConnectorPlacement.EquallySpacedConnector\",\"uuid\":\"1bda90bf-7ec8-4676-b4c1-6df6810f307f\"}],\"packageUris\":[\"http://schema.mathworks.com/mf0/Connector/R2020b\"],\"version\":\"1.0\"}"
  Navigation & State Estimation : Subsystem
      settings: PortSchema="{\"entries\":[{\"content\":{\"headerSize\":26,\"margin\":15,\"minimumSpacing\":25,\"sides\":[{\"content\":{\"connectorIds\":[\"In1\",\"In2\"]},\"type\":\"ConnectorPlacement.EquallySpacedRectSide\",\"uuid\":\"bfc9b5ca-65d3-4883-965c-09cadc06ae86\"},{\"content\":{\"connectorIds\":[\"Out1\",\"Out2\",\"Out3\",\"Out4\"],\"side\":\"RIGHT\"},\"type\":\"ConnectorPlacement.EquallySpacedRectSide\",\"uuid\":\"302eddba-73e5-4bab-ba05-7a4cd66d036f\"},{\"content\":{\"side\":\"TOP\"},\"type\":\"ConnectorPlacement.EquallySpacedRectSide\",\"uuid\":\"ad98d540-1dfa-45ea-9ded-5f35e32eb634\"}]},\"type\":\"ConnectorPlacement.EquallySpacedConnector\",\"uuid\":\"1bda90bf-7ec8-4676-b4c1-6df6810f307f\"}],\"packageUris\":[\"http://schema.mathworks.com/mf0/Connector/R2020b\"],\"version\":\"1.0\"}"
  IF-PWR-GNC-01 : PMIOPort  Side=Left  ConnectionType=Bus: ElectricalPower
  Bus Element Out5 : Outport  PortName=IF-GNC-ACT-01
  Bus Element Out1 : Outport  Port=2  PortName=IF-GNC-BEC-01
  Bus Element Out2 : Outport  Port=3  PortName=IF-GNC-SEC-01
  Bus Element Out3 : Outport  Port=4  PortName=IF-GNC-TVC-01
  Bus Element Out4 : Outport  Port=5  PortName=IF-GNC-RCT-01
  Bus Element Out6 : Outport  Port=6  PortName=IF-GNC-BFC-01
  Bus Element Out7 : Outport  Port=7  PortName=IF-GNC-SFC-01
  Bus Element Out8 : Outport  Port=8  PortName=IF-GNC-BPR-01
  Bus Element Out9 : Outport  Port=9  PortName=IF-GNC-SPR-01
  Bus Element Out10 : Outport  Port=10  PortName=IF-GNC-BTA-01
  Bus Element Out11 : Outport  Port=11  PortName=IF-GNC-STA-01
  Bus Element Out12 : Outport  Port=12  PortName=IF-GNC-TMS-01
  Bus Element Out13 : Outport  Port=13  PortName=IF-FHM-SAF-01
  wires:
  Control Command & Allocation/4(IF-GNC-BFC-01) -> Bus Element Out6/1
  Guidance & Trajectory Management/2(IF-GPH-CTR-01) -> Flight Control/2(IF-GPH-CTR-01)
  Bus Element In4/1 -> Navigation & State Estimation/2(IF-TMS-GNC-01)
  Navigation & State Estimation/3(IF-NSE-CAT-01) -> Flight Control/4(IF-NSE-CAT-01)
  Navigation & State Estimation/1(IF-NSE-GPH-01) -> Guidance & Trajectory Management/1(IF-NSE-GPH-01)
  Navigation & State Estimation/4(IF-NVI-FHM-01) -> GNC Flight Software & Mode Management/5(IF-NVI-FHM-01)
  Navigation & State Estimation/2(IF-NSE-CTR-01) -> Flight Control/3(IF-NSE-CTR-01)
  Guidance & Trajectory Management/1(IF-GPH-CAT-01) -> Flight Control/1(IF-GPH-CAT-01)
  GNC Flight Software & Mode Management/1(IF-GNC-TMS-01) -> Bus Element Out12/1
  GNC Flight Software & Mode Management/2(IF-GNC-STA-01) -> Bus Element Out11/1
  GNC Flight Software & Mode Management/3(IF-GNC-BTA-01) -> Bus Element Out10/1
  GNC Flight Software & Mode Management/4(IF-FMG-GMD-01) -> Guidance & Trajectory Management/2(IF-FMG-GMD-01)
  GNC Flight Software & Mode Management/5(IF-FMG-CAM-01) -> Flight Control/5(IF-FMG-CAM-01)
  Flight Control/1(IF-CLM-CAS-01) -> Control Command & Allocation/1(IF-CLM-CAS-01)
  Control Command & Allocation/1(IF-GNC-SPR-01) -> Bus Element Out9/1
  Control Command & Allocation/2(IF-GNC-BPR-01) -> Bus Element Out8/1
  Control Command & Allocation/3(IF-GNC-SFC-01) -> Bus Element Out7/1
  Control Command & Allocation/5(IF-GNC-RCT-01) -> Bus Element Out4/1
  Control Command & Allocation/6(IF-GNC-TVC-01) -> Bus Element Out3/1
  Control Command & Allocation/7(IF-GNC-SEC-01) -> Bus Element Out2/1
  Control Command & Allocation/8(IF-GNC-BEC-01) -> Bus Element Out1/1
  Control Command & Allocation/9(IF-CRS-FHM-01) -> GNC Flight Software & Mode Management/6(IF-CRS-FHM-01)
  Control Command & Allocation/10(IF-GNC-ACT-01) -> Bus Element Out5/1
  Bus Element In5/1 -> Navigation & State Estimation/1(IF-POS-GNC-01)
  Bus Element In1/1 -> GNC Flight Software & Mode Management/4(IF-TVC-GNC-01)
  Bus Element In2/1 -> GNC Flight Software & Mode Management/3(IF-BCR-GNC-01)
  Bus Element In3/1 -> GNC Flight Software & Mode Management/2(IF-SCR-GNC-01)
  GNC Flight Software & Mode Management/6(IF-FHM-SAF-01) -> Bus Element Out13/1
  Bus Element In6/1 -> GNC Flight Software & Mode Management/1(IF-SAF-FHM-01)
  connections:
  IF-PWR-GNC-01/RConn1 -- Control Command & Allocation/LConn1

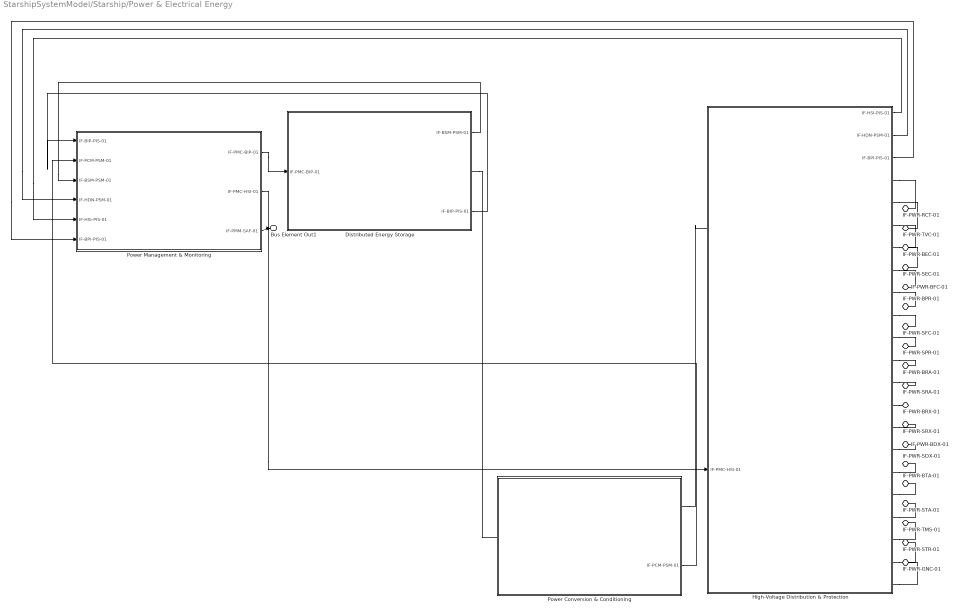
== system StarshipSystemModel/Starship/Power & Electrical Energy ==
  Distributed Energy Storage : Subsystem
      settings: PortSchema="{\"entries\":[{\"content\":{\"headerSize\":26,\"margin\":15,\"minimumSpacing\":25,\"sides\":[{\"content\":{\"connectorIds\":[\"In1\"]},\"type\":\"ConnectorPlacement.EquallySpacedRectSide\",\"uuid\":\"e231466c-79f3-4a10-9258-08b328dbb315\"},{\"content\":{\"connectorIds\":[\"Out1\",\"RConn1\",\"Out2\"],\"side\":\"RIGHT\"},\"type\":\"ConnectorPlacement.EquallySpacedRectSide\",\"uuid\":\"d7277c0a-5b77-426a-ad5b-7f06851f857a\"},{\"content\":{\"side\":\"TOP\"},\"type\":\"ConnectorPlacement.EquallySpacedRectSide\",\"uuid\":\"72d60576-32e4-4fd9-b552-a617024da2ce\"}]},\"type\":\"ConnectorPlacement.EquallySpacedConnector\",\"uuid\":\"6309e805-37c0-4868-97b0-5f8fd0bed587\"}],\"packageUris\":[\"http://schema.mathworks.com/mf0/Connector/R2020b\"],\"version\":\"1.0\"}"
  High-Voltage Distribution & Protection : Subsystem
      settings: PortSchema="{\"entries\":[{\"content\":{\"headerSize\":26,\"margin\":15,\"minimumSpacing\":25,\"sides\":[{\"content\":{\"connectorIds\":[\"LConn1\",\"In1\"]},\"type\":\"ConnectorPlacement.EquallySpacedRectSide\",\"uuid\":\"e231466c-79f3-4a10-9258-08b328dbb315\"},{\"content\":{\"connectorIds\":[\"Out2\",\"Out3\",\"Out1\",\"RConn1\",\"RConn2\",\"RConn3\",\"RConn4\",\"RConn5\",\"RConn6\",\"RConn7\",\"RConn8\",\"RConn9\",\"RConn10\",\"RConn11\",\"RConn12\",\"RConn13\",\"RConn14\",\"RConn15\",\"RConn16\",\"RConn17\",\"RConn18\",\"RConn19\"],\"side\":\"RIGHT\"},\"type\":\"ConnectorPlacement.EquallySpacedRectSide\",\"uuid\":\"d7277c0a-5b77-426a-ad5b-7f06851f857a\"},{\"content\":{\"side\":\"TOP\"},\"type\":\"ConnectorPlacement.EquallySpacedRectSide\",\"uuid\":\"72d60576-32e4-4fd9-b552-a617024da2ce\"}]},\"type\":\"ConnectorPlacement.EquallySpacedConnector\",\"uuid\":\"6309e805-37c0-4868-97b0-5f8fd0bed587\"}],\"packageUris\":[\"http://schema.mathworks.com/mf0/Connector/R2020b\"],\"version\":\"1.0\"}"
  Power Conversion & Conditioning : Subsystem
      settings: PortSchema="{\"entries\":[{\"content\":{\"headerSize\":26,\"margin\":15,\"minimumSpacing\":25,\"sides\":[{\"content\":{\"connectorIds\":[\"LConn1\"]},\"type\":\"ConnectorPlacement.EquallySpacedRectSide\",\"uuid\":\"e231466c-79f3-4a10-9258-08b328dbb315\"},{\"content\":{\"connectorIds\":[\"RConn1\",\"Out1\"],\"side\":\"RIGHT\"},\"type\":\"ConnectorPlacement.EquallySpacedRectSide\",\"uuid\":\"d7277c0a-5b77-426a-ad5b-7f06851f857a\"},{\"content\":{\"side\":\"TOP\"},\"type\":\"ConnectorPlacement.EquallySpacedRectSide\",\"uuid\":\"72d60576-32e4-4fd9-b552-a617024da2ce\"}]},\"type\":\"ConnectorPlacement.EquallySpacedConnector\",\"uuid\":\"6309e805-37c0-4868-97b0-5f8fd0bed587\"}],\"packageUris\":[\"http://schema.mathworks.com/mf0/Connector/R2020b\"],\"version\":\"1.0\"}"
  Power Management & Monitoring : Subsystem
      settings: PortSchema="{\"entries\":[{\"content\":{\"headerSize\":26,\"margin\":15,\"minimumSpacing\":25,\"sides\":[{\"content\":{\"connectorIds\":[\"In1\",\"In2\",\"In3\",\"In4\",\"In5\",\"In6\"]},\"type\":\"ConnectorPlacement.EquallySpacedRectSide\",\"uuid\":\"e231466c-79f3-4a10-9258-08b328dbb315\"},{\"content\":{\"connectorIds\":[\"Out1\",\"Out2\",\"Out3\"],\"side\":\"RIGHT\"},\"type\":\"ConnectorPlacement.EquallySpacedRectSide\",\"uuid\":\"d7277c0a-5b77-426a-ad5b-7f06851f857a\"},{\"content\":{\"side\":\"TOP\"},\"type\":\"ConnectorPlacement.EquallySpacedRectSide\",\"uuid\":\"72d60576-32e4-4fd9-b552-a617024da2ce\"}]},\"type\":\"ConnectorPlacement.EquallySpacedConnector\",\"uuid\":\"6309e805-37c0-4868-97b0-5f8fd0bed587\"}],\"packageUris\":[\"http://schema.mathworks.com/mf0/Connector/R2020b\"],\"version\":\"1.0\"}"
  IF-PWR-RCT-01 : PMIOPort  Side=Right  ConnectionType=Bus: ElectricalPower
  IF-PWR-TVC-01 : PMIOPort  Port=2  Side=Right  ConnectionType=Bus: ElectricalPower
  IF-PWR-BEC-01 : PMIOPort  Port=3  Side=Right  ConnectionType=Bus: ElectricalPower
  IF-PWR-SEC-01 : PMIOPort  Port=4  Side=Right  ConnectionType=Bus: ElectricalPower
  IF-PWR-BPR-01 : PMIOPort  Port=5  Side=Right  ConnectionType=Bus: ElectricalPower
  IF-PWR-BFC-01 : PMIOPort  Port=6  Side=Right  ConnectionType=Bus: ElectricalPower
  IF-PWR-SFC-01 : PMIOPort  Port=7  Side=Right  ConnectionType=Bus: ElectricalPower
  IF-PWR-SPR-01 : PMIOPort  Port=8  Side=Right  ConnectionType=Bus: ElectricalPower
  IF-PWR-BRA-01 : PMIOPort  Port=9  Side=Right  ConnectionType=Bus: ElectricalPower
  IF-PWR-SRA-01 : PMIOPort  Port=10  Side=Right  ConnectionType=Bus: ElectricalPower
  IF-PWR-BRX-01 : PMIOPort  Port=11  Side=Right  ConnectionType=Bus: ElectricalPower
  IF-PWR-SRX-01 : PMIOPort  Port=12  Side=Right  ConnectionType=Bus: ElectricalPower
  IF-PWR-BDX-01 : PMIOPort  Port=13  Side=Right  ConnectionType=Bus: ElectricalPower
  IF-PWR-SDX-01 : PMIOPort  Port=14  Side=Right  ConnectionType=Bus: ElectricalPower
  IF-PWR-BTA-01 : PMIOPort  Port=15  Side=Right  ConnectionType=Bus: ElectricalPower
  IF-PWR-STA-01 : PMIOPort  Port=16  Side=Right  ConnectionType=Bus: ElectricalPower
  IF-PWR-TMS-01 : PMIOPort  Port=17  Side=Right  ConnectionType=Bus: ElectricalPower
  IF-PWR-STR-01 : PMIOPort  Port=18  Side=Right  ConnectionType=Bus: ElectricalPower
  IF-PWR-GNC-01 : PMIOPort  Port=19  Side=Right  ConnectionType=Bus: ElectricalPower
  Bus Element Out1 : Outport  PortName=IF-PMM-SAF-01
  wires:
  Distributed Energy Storage/1(IF-BSM-PSM-01) -> Power Management & Monitoring/3(IF-BSM-PSM-01)
  High-Voltage Distribution & Protection/2(IF-HSI-PIS-01) -> Power Management & Monitoring/5(IF-HSI-PIS-01)
  High-Voltage Distribution & Protection/1(IF-BPI-PIS-01) -> Power Management & Monitoring/6(IF-BPI-PIS-01)
  Power Conversion & Conditioning/1(IF-PCM-PSM-01) -> Power Management & Monitoring/2(IF-PCM-PSM-01)
  Distributed Energy Storage/2(IF-BIP-PIS-01) -> Power Management & Monitoring/1(IF-BIP-PIS-01)
  High-Voltage Distribution & Protection/3(IF-HDN-PSM-01) -> Power Management & Monitoring/4(IF-HDN-PSM-01)
  Power Management & Monitoring/1(IF-PMC-BIP-01) -> Distributed Energy Storage/1(IF-PMC-BIP-01)
  Power Management & Monitoring/2(IF-PMC-HSI-01) -> High-Voltage Distribution & Protection/1(IF-PMC-HSI-01)
  Power Management & Monitoring/3(IF-PMM-SAF-01) -> Bus Element Out1/1
  connections:
  High-Voltage Distribution & Protection/RConn16 -- IF-PWR-STA-01/RConn1
  High-Voltage Distribution & Protection/RConn18 -- IF-PWR-STR-01/RConn1
  High-Voltage Distribution & Protection/RConn17 -- IF-PWR-TMS-01/RConn1
  Distributed Energy Storage/RConn1 -- Power Conversion & Conditioning/LConn1
  Power Conversion & Conditioning/RConn1 -- High-Voltage Distribution & Protection/LConn1
  High-Voltage Distribution & Protection/RConn1 -- IF-PWR-RCT-01/RConn1
  High-Voltage Distribution & Protection/RConn2 -- IF-PWR-TVC-01/RConn1
  High-Voltage Distribution & Protection/RConn3 -- IF-PWR-BEC-01/RConn1
  High-Voltage Distribution & Protection/RConn4 -- IF-PWR-SEC-01/RConn1
  High-Voltage Distribution & Protection/RConn5 -- IF-PWR-BFC-01/RConn1
  High-Voltage Distribution & Protection/RConn6 -- IF-PWR-BPR-01/RConn1
  High-Voltage Distribution & Protection/RConn7 -- IF-PWR-SFC-01/RConn1
  High-Voltage Distribution & Protection/RConn8 -- IF-PWR-SPR-01/RConn1
  High-Voltage Distribution & Protection/RConn9 -- IF-PWR-BRA-01/RConn1
  High-Voltage Distribution & Protection/RConn10 -- IF-PWR-SRA-01/RConn1
  High-Voltage Distribution & Protection/RConn11 -- IF-PWR-BRX-01/RConn1
  High-Voltage Distribution & Protection/RConn12 -- IF-PWR-SRX-01/RConn1
  High-Voltage Distribution & Protection/RConn13 -- IF-PWR-BDX-01/RConn1
  High-Voltage Distribution & Protection/RConn14 -- IF-PWR-SDX-01/RConn1
  High-Voltage Distribution & Protection/RConn15 -- IF-PWR-BTA-01/RConn1
  High-Voltage Distribution & Protection/RConn19 -- IF-PWR-GNC-01/RConn1
